simulink model "rfsoc4x2_ospfb_128"  (R2021a)
(part 2 of 221)

      mask Callback t224_QT_adc3_enable: enable_adc_opt(gcb,224,3,'QT');
      mask TypeOptions t224_QT_adc3_digital_output: Real | I/Q
      mask Callback t224_QT_adc3_digital_output:
      | validate_digital_data(gcb,224,3,'QT');
      | update_axis_clk(gcb,224);
      mask TypeOptions t224_QT_adc3_dec_mode: 1x | 2x | 3x | 4x | 5x | 6x | 8x | 10x | 12x | 16x | 20x | 24x | 40x
      mask Callback t224_QT_adc3_dec_mode: update_axis_clk(gcb,224);
      mask TypeOptions t224_QT_adc3_sample_per_cycle: 4 | 5 | 6 | 7 | 8 | 9 | 10 | 11 | 12
      mask Callback t224_QT_adc3_sample_per_cycle: update_axis_clk_label(gcb,224);
      mask TypeOptions t224_QT_adc3_mixer_type: Bypassed
      mask Callback t224_QT_adc3_mixer_type: mixertype_callback(gcb,224,3,'QT');
      mask TypeOptions t224_QT_adc3_mixer_mode: Real -> Real
      mask Callback t224_QT_adc3_mixer_mode: mixer_callback(gcb,224,3,'QT')
      mask TypeOptions t224_QT_adc3_coarse_freq: 0
      mask TypeOptions t224_QT_adc3_nyquist_zone: Zone 1 | Zone 2
      mask TypeOptions t224_QT_adc3_cal_mode: Mode 1 | Mode 2
      mask Callback t224_DT_adc0_enable: enable_adc_opt(gcb,224,0,'DT');
      mask TypeOptions t224_DT_adc0_digital_output: Real | I/Q
      mask Callback t224_DT_adc0_digital_output:
      | validate_digital_data(gcb,224,0,'DT');
      | update_axis_clk(gcb,224);
      mask TypeOptions t224_DT_adc0_dec_mode: 1x | 2x | 3x | 4x | 5x | 6x | 8x | 10x | 12x | 16x | 20x | 24x | 40x
      mask Callback t224_DT_adc0_dec_mode:
      | % if I/Q output mode, need to copy interp factor before updating axis clk
      | % note only the even slice for the tile makes this check
      | if chk_param(gcb, 't224_DT_adc0_mixer_mode', 'I/Q -> I/Q')
      |   dec_mode = get_param(gcb, 't224_DT_adc0_dec_mode');
      |   set_param(gcb, 't224_DT_adc1_dec_mode', dec_mode);
      | end
      | 
      | update_axis_clk(gcb,224);
      mask TypeOptions t224_DT_adc0_sample_per_cycle: 4 | 5 | 6 | 7 | 8 | 9 | 10 | 11 | 12
      mask Callback t224_DT_adc0_sample_per_cycle:
      | % if I/Q output mode, need to copy samples per clk before updating axis clk
      | % note only the even slice for the tile makes this check
      | if chk_param(gcb, 't224_DT_adc0_mixer_mode', 'I/Q -> I/Q')
      |   spc = get_param(gcb, 't224_DT_adc0_sample_per_cycle');
      |   set_param(gcb, 't224_DT_adc1_sample_per_cycle', spc);
      | end
      | update_axis_clk_label(gcb,224);
      mask TypeOptions t224_DT_adc0_mixer_type: Bypassed
      mask Callback t224_DT_adc0_mixer_type: mixertype_callback(gcb,224,0,'DT');
      mask TypeOptions t224_DT_adc0_mixer_mode: Real -> Real
      mask Callback t224_DT_adc0_mixer_mode: mixer_callback(gcb,224,0,'DT');
      mask TypeOptions t224_DT_adc0_coarse_freq: 0
      mask TypeOptions t224_DT_adc0_nyquist_zone: Zone 1 | Zone 2
      mask TypeOptions t224_DT_adc0_cal_mode: Mode 1 | Mode 2
      mask Callback t224_DT_adc1_enable: enable_adc_opt(gcb,224,1,'DT');
      mask TypeOptions t224_DT_adc1_digital_output: Real | I/Q
      mask Callback t224_DT_adc1_digital_output:
      | validate_digital_data(gcb,224,1,'DT');
      | update_axis_clk(gcb,224);
      mask TypeOptions t224_DT_adc1_dec_mode: 1x | 2x | 3x | 4x | 5x | 6x | 8x | 10x | 12x | 16x | 20x | 24x | 40x
      mask Callback t224_DT_adc1_dec_mode: update_axis_clk(gcb,224);
      mask TypeOptions t224_DT_adc1_sample_per_cycle: 4 | 5 | 6 | 7 | 8 | 9 | 10 | 11 | 12
      mask Callback t224_DT_adc1_sample_per_cycle:
      | %update_axis_clk(gcb);
      | update_axis_clk_label(gcb,224);
      mask TypeOptions t224_DT_adc1_mixer_type: Bypassed
      mask Callback t224_DT_adc1_mixer_type: mixertype_callback(gcb,224,1,'DT');
      mask TypeOptions t224_DT_adc1_mixer_mode: Real -> Real
      mask Callback t224_DT_adc1_mixer_mode: mixer_callback(gcb,224,1,'DT');
      mask TypeOptions t224_DT_adc1_coarse_freq: 0
      mask TypeOptions t224_DT_adc1_nyquist_zone: Zone 1 | Zone 2
      mask TypeOptions t224_DT_adc1_cal_mode: Mode 1 | Mode 2
      mask Callback t225_sample_rate: update_rfdc_clocking(gcb,225);
      mask TypeOptions t225_clk_out: 100 | 50 | 25 | 12.5
      mask Callback t225_enable_pll:
      | %update_rfdc_clocking(gcb);
      | update_pll(gcb,225);
      mask TypeOptions t225_ref_clk: 738.462 | 685.714 | 640 | 600 | 564.706 | 533.333 | 505.263 | 480 | 457.143 | 436.364 | 417.391 | 400 | 384 | 369.231 | 355.556 | 342.857 | 331.034 | 320 | 309.677 | 300 | 290.909 | 282.353 | 274.286 | 266.667 | 259.459 | 252.632 | 246.154 | 240 | 234.146 | 228.571 | 223.256 | 218.182 | 213.333 | 208.696 | 204.255 | 200 | 195.918 | 192 | 188.235 | 184.615 | 181.132 | 177.778 | 174.545 | 171.429 | 168.421 | 165.517 | 162.712 | 160 | 157.377 | 154.839 | 152.381 | 150 | 147.692 | 145.455 | 143.284 | 141.176 | 139.13 | 137.143 | 135.211 | 133.333 | 131.507 | 129.73 | 128 | 126.316 | 124.675 | 123.077 | 121.519 | 120 | 118.519 | 117.073 | 115.663 | 114.286 | 112.941 | 111.628 | 110.345 | 109.091 | 107.865 | 106.667 | 105.495 | 104.348 | 103.226
      mask Callback t225_QT_adc0_enable: enable_adc_opt(gcb,225,0,'QT');
      mask TypeOptions t225_QT_adc0_digital_output: Real | I/Q
      mask Callback t225_QT_adc0_digital_output:
      | validate_digital_data(gcb,225,0,'QT');
      | update_axis_clk(gcb,225);
      mask TypeOptions t225_QT_adc0_dec_mode: 1x | 2x | 3x | 4x | 5x | 6x | 8x | 10x | 12x | 16x | 20x | 24x | 40x
      mask Callback t225_QT_adc0_dec_mode:
      | % if I/Q output mode, need to copy interp factor before updating axis clk
      | % note only the even slice for the tile makes this check
      | if chk_param(gcb, 't225_QT_adc0_mixer_mode', 'I/Q -> I/Q')
      |   dec_mode = get_param(gcb, 't225_QT_adc0_dec_mode');
      |   set_param(gcb, 't225_QT_adc1_dec_mode', dec_mode);
      | end
      | update_axis_clk(gcb,225);
      mask TypeOptions t225_QT_adc0_sample_per_cycle: 4 | 5 | 6 | 7 | 8 | 9 | 10 | 11 | 12
      mask Callback t225_QT_adc0_sample_per_cycle:
      | % if I/Q output mode, need to copy samples per clk before updating axis clk
      | % note only the even slice for the tile makes this check
      | if chk_param(gcb, 't225_QT_adc0_mixer_mode', 'I/Q -> I/Q')
      |   spc = get_param(gcb, 't225_QT_adc0_sample_per_cycle');
      |   set_param(gcb, 't225_QT_adc1_sample_per_cycle', spc);
      | end
      | update_axis_clk_label(gcb,225);
      mask TypeOptions t225_QT_adc0_mixer_type: Bypassed
      mask Callback t225_QT_adc0_mixer_type: mixertype_callback(gcb,225,0,'QT');
      mask TypeOptions t225_QT_adc0_mixer_mode: Real -> Real
      mask Callback t225_QT_adc0_mixer_mode: mixer_callback(gcb,225,0,'QT');
      mask TypeOptions t225_QT_adc0_coarse_freq: 0
      mask TypeOptions t225_QT_adc0_nyquist_zone: Zone 1 | Zone 2
      mask TypeOptions t225_QT_adc0_cal_mode: Mode 1 | Mode 2
      mask Callback t225_QT_adc1_enable: enable_adc_opt(gcb,225,1,'QT');
      mask TypeOptions t225_QT_adc1_digital_output: Real | I/Q
      mask Callback t225_QT_adc1_digital_output:
      | validate_digital_data(gcb,225,1,'QT');
      | update_axis_clk(gcb,225);
      mask TypeOptions t225_QT_adc1_dec_mode: 1x | 2x | 3x | 4x | 5x | 6x | 8x | 10x | 12x | 16x | 20x | 24x | 40x
      mask Callback t225_QT_adc1_dec_mode: update_axis_clk(gcb,225);
      mask TypeOptions t225_QT_adc1_sample_per_cycle: 4 | 5 | 6 | 7 | 8 | 9 | 10 | 11 | 12
      mask Callback t225_QT_adc1_sample_per_cycle: update_axis_clk_label(gcb,225);
      mask TypeOptions t225_QT_adc1_mixer_type: Bypassed
      mask Callback t225_QT_adc1_mixer_type: mixertype_callback(gcb,225,1,'QT');
      mask TypeOptions t225_QT_adc1_mixer_mode: Real -> Real
      mask Callback t225_QT_adc1_mixer_mode: mixer_callback(gcb,225,1,'QT')
      mask TypeOptions t225_QT_adc1_coarse_freq: 0
      mask TypeOptions t225_QT_adc1_nyquist_zone: Zone 1 | Zone 2
      mask TypeOptions t225_QT_adc1_cal_mode: Mode 1 | Mode 2
      mask Callback t225_QT_adc2_enable: enable_adc_opt(gcb,225,2,'QT');
      mask TypeOptions t225_QT_adc2_digital_output: Real | I/Q
      mask Callback t225_QT_adc2_digital_output:
      | validate_digital_data(gcb,225,2,'QT');
      | update_axis_clk(gcb,225);
      mask TypeOptions t225_QT_adc2_dec_mode: 1x | 2x | 3x | 4x | 5x | 6x | 8x | 10x | 12x | 16x | 20x | 24x | 40x
      mask Callback t225_QT_adc2_dec_mode:
      | % if I/Q output mode, need to copy interp factor before updating axis clk
      | % note only the even slice for the tile makes this check
      | if chk_param(gcb, 't225_QT_adc2_mixer_mode', 'I/Q -> I/Q')
      |   dec_mode = get_param(gcb, 't225_QT_adc2_dec_mode');
      |   set_param(gcb, 't225_QT_adc3_dec_mode', dec_mode);
      | end
      | update_axis_clk(gcb,225);
      mask TypeOptions t225_QT_adc2_sample_per_cycle: 4 | 5 | 6 | 7 | 8 | 9 | 10 | 11 | 12
      mask Callback t225_QT_adc2_sample_per_cycle:
      | % if I/Q output mode, need to copy samples per clk before updating axis clk
      | % note only the even slice for the tile makes this check
      | if chk_param(gcb, 't225_QT_adc2_mixer_mode', 'I/Q -> I/Q')
      |   spc = get_param(gcb, 't225_QT_adc2_sample_per_cycle');
      |   set_param(gcb, 't225_QT_adc3_sample_per_cycle', spc);
      | end
      | update_axis_clk_label(gcb,225);
      mask TypeOptions t225_QT_adc2_mixer_type: Bypassed
      mask Callback t225_QT_adc2_mixer_type: mixertype_callback(gcb,225,2,'QT');
      mask TypeOptions t225_QT_adc2_mixer_mode: Real -> Real
      mask Callback t225_QT_adc2_mixer_mode: mixer_callback(gcb,225,2,'QT')
      mask TypeOptions t225_QT_adc2_coarse_freq: 0
      mask TypeOptions t225_QT_adc2_nyquist_zone: Zone 1 | Zone 2
      mask TypeOptions t225_QT_adc2_cal_mode: Mode 1 | Mode 2
      mask Callback t225_QT_adc3_enable: enable_adc_opt(gcb,225,3,'QT');
      mask TypeOptions t225_QT_adc3_digital_output: Real | I/Q
      mask Callback t225_QT_adc3_digital_output:
      | validate_digital_data(gcb,225,3,'QT');
      | update_axis_clk(gcb,225);
      mask TypeOptions t225_QT_adc3_dec_mode: 1x | 2x | 3x | 4x | 5x | 6x | 8x | 10x | 12x | 16x | 20x | 24x | 40x
      mask Callback t225_QT_adc3_dec_mode: update_axis_clk(gcb,225);
      mask TypeOptions t225_QT_adc3_sample_per_cycle: 4 | 5 | 6 | 7 | 8 | 9 | 10 | 11 | 12
      mask Callback t225_QT_adc3_sample_per_cycle: update_axis_clk_label(gcb,225);
      mask TypeOptions t225_QT_adc3_mixer_type: Bypassed
      mask Callback t225_QT_adc3_mixer_type: mixertype_callback(gcb,225,3,'QT');
      mask TypeOptions t225_QT_adc3_mixer_mode: Real -> Real
      mask Callback t225_QT_adc3_mixer_mode: mixer_callback(gcb,225,3,'QT')
      mask TypeOptions t225_QT_adc3_coarse_freq: 0
      mask TypeOptions t225_QT_adc3_nyquist_zone: Zone 1 | Zone 2
      mask TypeOptions t225_QT_adc3_cal_mode: Mode 1 | Mode 2
      mask Callback t225_DT_adc0_enable: enable_adc_opt(gcb,225,0,'DT');
      mask TypeOptions t225_DT_adc0_digital_output: Real | I/Q
      mask Callback t225_DT_adc0_digital_output:
      | validate_digital_data(gcb,225,0,'DT');
      | update_axis_clk(gcb,225);
      mask TypeOptions t225_DT_adc0_dec_mode: 1x | 2x | 3x | 4x | 5x | 6x | 8x | 10x | 12x | 16x | 20x | 24x | 40x
      mask Callback t225_DT_adc0_dec_mode:
      | % if I/Q output mode, need to copy interp factor before updating axis clk
      | % note only the even slice for the tile makes this check
      | if chk_param(gcb, 't225_DT_adc0_mixer_mode', 'I/Q -> I/Q')
      |   dec_mode = get_param(gcb, 't225_DT_adc0_dec_mode');
      |   set_param(gcb, 't225_DT_adc1_dec_mode', dec_mode);
      | end
      | update_axis_clk(gcb,225);
      mask TypeOptions t225_DT_adc0_sample_per_cycle: 4 | 5 | 6 | 7 | 8 | 9 | 10 | 11 | 12
      mask Callback t225_DT_adc0_sample_per_cycle:
      | % if I/Q output mode, need to copy samples per clk before updating axis clk
      | % note only the even slice for the tile makes this check
      | if chk_param(gcb, 't225_DT_adc0_mixer_mode', 'I/Q -> I/Q')
      |   spc = get_param(gcb, 't225_DT_adc0_sample_per_cycle');
      |   set_param(gcb, 't225_DT_adc1_sample_per_cycle', spc);
      | end
      | update_axis_clk_label(gcb,225);
      mask TypeOptions t225_DT_adc0_mixer_type: Bypassed
      mask Callback t225_DT_adc0_mixer_type: mixertype_callback(gcb,225,0,'DT');
      mask TypeOptions t225_DT_adc0_mixer_mode: Real -> Real
      mask Callback t225_DT_adc0_mixer_mode: mixer_callback(gcb,225,0,'DT');
      mask TypeOptions t225_DT_adc0_coarse_freq: 0
      mask TypeOptions t225_DT_adc0_nyquist_zone: Zone 1 | Zone 2
      mask TypeOptions t225_DT_adc0_cal_mode: Mode 1 | Mode 2
      mask Callback t225_DT_adc1_enable: enable_adc_opt(gcb,225,1,'DT');
      mask TypeOptions t225_DT_adc1_digital_output: Real | I/Q
      mask Callback t225_DT_adc1_digital_output:
      | validate_digital_data(gcb,225,1,'DT');
      | update_axis_clk(gcb,225);
      mask TypeOptions t225_DT_adc1_dec_mode: 1x | 2x | 3x | 4x | 5x | 6x | 8x | 10x | 12x | 16x | 20x | 24x | 40x
      mask Callback t225_DT_adc1_dec_mode: update_axis_clk(gcb,225);
      mask TypeOptions t225_DT_adc1_sample_per_cycle: 4 | 5 | 6 | 7 | 8 | 9 | 10 | 11 | 12
      mask Callback t225_DT_adc1_sample_per_cycle:
      | %update_axis_clk(gcb);
      | update_axis_clk_label(gcb,225);
      mask TypeOptions t225_DT_adc1_mixer_type: Bypassed
      mask Callback t225_DT_adc1_mixer_type: mixertype_callback(gcb,225,1,'DT');
      mask TypeOptions t225_DT_adc1_mixer_mode: Real -> Real
      mask Callback t225_DT_adc1_mixer_mode: mixer_callback(gcb,225,1,'DT');
      mask TypeOptions t225_DT_adc1_coarse_freq: 0
      mask TypeOptions t225_DT_adc1_nyquist_zone: Zone 1 | Zone 2
      mask TypeOptions t225_DT_adc1_cal_mode: Mode 1 | Mode 2
      mask Callback t226_sample_rate: update_rfdc_clocking(gcb,226);
      mask TypeOptions t226_clk_out: 100 | 50 | 25 | 12.5
      mask Callback t226_enable_pll:
      | %update_rfdc_clocking(gcb);
      | update_pll(gcb,226);
      mask TypeOptions t226_ref_clk: 738.462 | 685.714 | 640 | 600 | 564.706 | 533.333 | 505.263 | 480 | 457.143 | 436.364 | 417.391 | 400 | 384 | 369.231 | 355.556 | 342.857 | 331.034 | 320 | 309.677 | 300 | 290.909 | 282.353 | 274.286 | 266.667 | 259.459 | 252.632 | 246.154 | 240 | 234.146 | 228.571 | 223.256 | 218.182 | 213.333 | 208.696 | 204.255 | 200 | 195.918 | 192 | 188.235 | 184.615 | 181.132 | 177.778 | 174.545 | 171.429 | 168.421 | 165.517 | 162.712 | 160 | 157.377 | 154.839 | 152.381 | 150 | 147.692 | 145.455 | 143.284 | 141.176 | 139.13 | 137.143 | 135.211 | 133.333 | 131.507 | 129.73 | 128 | 126.316 | 124.675 | 123.077 | 121.519 | 120 | 118.519 | 117.073 | 115.663 | 114.286 | 112.941 | 111.628 | 110.345 | 109.091 | 107.865 | 106.667 | 105.495 | 104.348 | 103.226
      mask Callback t226_QT_adc0_enable: enable_adc_opt(gcb,226,0,'QT');
      mask TypeOptions t226_QT_adc0_digital_output: Real | I/Q
      mask Callback t226_QT_adc0_digital_output:
      | validate_digital_data(gcb,226,0,'QT');
      | update_axis_clk(gcb,226);
      mask TypeOptions t226_QT_adc0_dec_mode: 1x | 2x | 3x | 4x | 5x | 6x | 8x | 10x | 12x | 16x | 20x | 24x | 40x
      mask Callback t226_QT_adc0_dec_mode:
      | % if I/Q output mode, need to copy interp factor before updating axis clk
      | % note only the even slice for the tile makes this check
      | if chk_param(gcb, 't226_QT_adc0_mixer_mode', 'I/Q -> I/Q')
      |   dec_mode = get_param(gcb, 't226_QT_adc0_dec_mode');
      |   set_param(gcb, 't226_QT_adc1_dec_mode', dec_mode);
      | end
      | update_axis_clk(gcb,226);
      mask TypeOptions t226_QT_adc0_sample_per_cycle: 4 | 5 | 6 | 7 | 8 | 9 | 10 | 11 | 12
      mask Callback t226_QT_adc0_sample_per_cycle:
      | % if I/Q output mode, need to copy samples per clk before updating axis clk
      | % note only the even slice for the tile makes this check
      | if chk_param(gcb, 't226_QT_adc0_mixer_mode', 'I/Q -> I/Q')
      |   spc = get_param(gcb, 't226_QT_adc0_sample_per_cycle');
      |   set_param(gcb, 't226_QT_adc1_sample_per_cycle', spc);
      | end
      | update_axis_clk_label(gcb,226);
      mask TypeOptions t226_QT_adc0_mixer_type: Bypassed
      mask Callback t226_QT_adc0_mixer_type: mixertype_callback(gcb,226,0,'QT');
      mask TypeOptions t226_QT_adc0_mixer_mode: Real -> Real
      mask Callback t226_QT_adc0_mixer_mode: mixer_callback(gcb,226,0,'QT');
      mask TypeOptions t226_QT_adc0_coarse_freq: 0
      mask TypeOptions t226_QT_adc0_nyquist_zone: Zone 1 | Zone 2
      mask TypeOptions t226_QT_adc0_cal_mode: Mode 1 | Mode 2
      mask Callback t226_QT_adc1_enable: enable_adc_opt(gcb,226,1,'QT');
      mask TypeOptions t226_QT_adc1_digital_output: Real | I/Q
      mask Callback t226_QT_adc1_digital_output:
      | validate_digital_data(gcb,226,1,'QT');
      | update_axis_clk(gcb,226);
      mask TypeOptions t226_QT_adc1_dec_mode: 1x | 2x | 3x | 4x | 5x | 6x | 8x | 10x | 12x | 16x | 20x | 24x | 40x
      mask Callback t226_QT_adc1_dec_mode: update_axis_clk(gcb,226);
      mask TypeOptions t226_QT_adc1_sample_per_cycle: 4 | 5 | 6 | 7 | 8 | 9 | 10 | 11 | 12
      mask Callback t226_QT_adc1_sample_per_cycle: update_axis_clk_label(gcb,226);
      mask TypeOptions t226_QT_adc1_mixer_type: Bypassed
      mask Callback t226_QT_adc1_mixer_type: mixertype_callback(gcb,226,1,'QT');
      mask TypeOptions t226_QT_adc1_mixer_mode: Real -> Real
      mask Callback t226_QT_adc1_mixer_mode: mixer_callback(gcb,226,1,'QT')
      mask TypeOptions t226_QT_adc1_coarse_freq: 0
      mask TypeOptions t226_QT_adc1_nyquist_zone: Zone 1 | Zone 2
      mask TypeOptions t226_QT_adc1_cal_mode: Mode 1 | Mode 2
      mask Callback t226_QT_adc2_enable: enable_adc_opt(gcb,226,2,'QT');
      mask TypeOptions t226_QT_adc2_digital_output: Real | I/Q
      mask Callback t226_QT_adc2_digital_output:
      | validate_digital_data(gcb,226,2,'QT');
      | update_axis_clk(gcb,226);
      mask TypeOptions t226_QT_adc2_dec_mode: 1x | 2x | 3x | 4x | 5x | 6x | 8x | 10x | 12x | 16x | 20x | 24x | 40x
      mask Callback t226_QT_adc2_dec_mode:
      | % if I/Q output mode, need to copy interp factor before updating axis clk
      | % note only the even slice for the tile makes this check
      | if chk_param(gcb, 't226_QT_adc2_mixer_mode', 'I/Q -> I/Q')
      |   dec_mode = get_param(gcb, 't226_QT_adc2_dec_mode');
      |   set_param(gcb, 't226_QT_adc3_dec_mode', dec_mode);
      | end
      | update_axis_clk(gcb,226);
      mask TypeOptions t226_QT_adc2_sample_per_cycle: 4 | 5 | 6 | 7 | 8 | 9 | 10 | 11 | 12
      mask Callback t226_QT_adc2_sample_per_cycle:
      | % if I/Q output mode, need to copy samples per clk before updating axis clk
      | % note only the even slice for the tile makes this check
      | if chk_param(gcb, 't226_QT_adc2_mixer_mode', 'I/Q -> I/Q')
      |   spc = get_param(gcb, 't226_QT_adc2_sample_per_cycle');
      |   set_param(gcb, 't226_QT_adc3_sample_per_cycle', spc);
      | end
      | update_axis_clk_label(gcb,226);
      mask TypeOptions t226_QT_adc2_mixer_type: Bypassed
      mask Callback t226_QT_adc2_mixer_type: mixertype_callback(gcb,226,2,'QT');
      mask TypeOptions t226_QT_adc2_mixer_mode: Real -> Real
      mask Callback t226_QT_adc2_mixer_mode: mixer_callback(gcb,226,2,'QT')
      mask TypeOptions t226_QT_adc2_coarse_freq: 0
      mask TypeOptions t226_QT_adc2_nyquist_zone: Zone 1 | Zone 2
      mask TypeOptions t226_QT_adc2_cal_mode: Mode 1 | Mode 2
      mask Callback t226_QT_adc3_enable: enable_adc_opt(gcb,226,3,'QT');
      mask TypeOptions t226_QT_adc3_digital_output: Real | I/Q
      mask Callback t226_QT_adc3_digital_output:
      | validate_digital_data(gcb,226,3,'QT');
      | update_axis_clk(gcb,226);
      mask TypeOptions t226_QT_adc3_dec_mode: 1x | 2x | 3x | 4x | 5x | 6x | 8x | 10x | 12x | 16x | 20x | 24x | 40x
      mask Callback t226_QT_adc3_dec_mode: update_axis_clk(gcb,226);
      mask TypeOptions t226_QT_adc3_sample_per_cycle: 4 | 5 | 6 | 7 | 8 | 9 | 10 | 11 | 12
      mask Callback t226_QT_adc3_sample_per_cycle: update_axis_clk_label(gcb,226);
      mask TypeOptions t226_QT_adc3_mixer_type: Bypassed
      mask Callback t226_QT_adc3_mixer_type: mixertype_callback(gcb,226,3,'QT');
      mask TypeOptions t226_QT_adc3_mixer_mode: Real -> Real
      mask Callback t226_QT_adc3_mixer_mode: mixer_callback(gcb,226,3,'QT')
      mask TypeOptions t226_QT_adc3_coarse_freq: 0
      mask TypeOptions t226_QT_adc3_nyquist_zone: Zone 1 | Zone 2
      mask TypeOptions t226_QT_adc3_cal_mode: Mode 1 | Mode 2
      mask Callback t226_DT_adc0_enable: enable_adc_opt(gcb,226,0,'DT');
      mask TypeOptions t226_DT_adc0_digital_output: Real | I/Q
      mask Callback t226_DT_adc0_digital_output:
      | validate_digital_data(gcb,226,0,'DT');
      | update_axis_clk(gcb,226);
      mask TypeOptions t226_DT_adc0_dec_mode: 1x | 2x | 3x | 4x | 5x | 6x | 8x | 10x | 12x | 16x | 20x | 24x | 40x
      mask Callback t226_DT_adc0_dec_mode:
      | % if I/Q output mode, need to copy interp factor before updating axis clk
      | % note only the even slice for the tile makes this check
      | if chk_param(gcb, 't226_DT_adc0_mixer_mode', 'I/Q -> I/Q')
      |   dec_mode = get_param(gcb, 't226_DT_adc0_dec_mode');
      |   set_param(gcb, 't226_DT_adc1_dec_mode', dec_mode);
      | end
      | update_axis_clk(gcb,226);
      mask TypeOptions t226_DT_adc0_sample_per_cycle: 4 | 5 | 6 | 7 | 8 | 9 | 10 | 11 | 12
      mask Callback t226_DT_adc0_sample_per_cycle:
      | % if I/Q output mode, need to copy samples per clk before updating axis clk
      | % note only the even slice for the tile makes this check
      | if chk_param(gcb, 't226_DT_adc0_mixer_mode', 'I/Q -> I/Q')
      |   spc = get_param(gcb, 't226_DT_adc0_sample_per_cycle');
      |   set_param(gcb, 't226_DT_adc1_sample_per_cycle', spc);
      | end
      | update_axis_clk_label(gcb,226);
      mask TypeOptions t226_DT_adc0_mixer_type: Bypassed
      mask Callback t226_DT_adc0_mixer_type: mixertype_callback(gcb,226,0,'DT');
      mask TypeOptions t226_DT_adc0_mixer_mode: Real -> Real
      mask Callback t226_DT_adc0_mixer_mode: mixer_callback(gcb,226,0,'DT');
      mask TypeOptions t226_DT_adc0_coarse_freq: 0
      mask TypeOptions t226_DT_adc0_nyquist_zone: Zone 1 | Zone 2
      mask TypeOptions t226_DT_adc0_cal_mode: Mode 1 | Mode 2
      mask Callback t226_DT_adc1_enable: enable_adc_opt(gcb,226,1,'DT');
      mask TypeOptions t226_DT_adc1_digital_output: Real | I/Q
      mask Callback t226_DT_adc1_digital_output:
      | validate_digital_data(gcb,226,1,'DT');
      | update_axis_clk(gcb,226);
      mask TypeOptions t226_DT_adc1_dec_mode: 1x | 2x | 3x | 4x | 5x | 6x | 8x | 10x | 12x | 16x | 20x | 24x | 40x
      mask Callback t226_DT_adc1_dec_mode: update_axis_clk(gcb,226);
      mask TypeOptions t226_DT_adc1_sample_per_cycle: 4 | 5 | 6 | 7 | 8 | 9 | 10 | 11 | 12
      mask Callback t226_DT_adc1_sample_per_cycle:
      | %update_axis_clk(gcb);
      | update_axis_clk_label(gcb,226);
      mask TypeOptions t226_DT_adc1_mixer_type: Bypassed
      mask Callback t226_DT_adc1_mixer_type: mixertype_callback(gcb,226,1,'DT');
      mask TypeOptions t226_DT_adc1_mixer_mode: Real -> Real
      mask Callback t226_DT_adc1_mixer_mode: mixer_callback(gcb,226,1,'DT');
      mask TypeOptions t226_DT_adc1_coarse_freq: 0
      mask TypeOptions t226_DT_adc1_nyquist_zone: Zone 1 | Zone 2
      mask TypeOptions t226_DT_adc1_cal_mode: Mode 1 | Mode 2
      mask Callback t227_sample_rate: update_rfdc_clocking(gcb,227);
      mask TypeOptions t227_clk_out: 100 | 50 | 25 | 12.5
      mask Callback t227_enable_pll:
      | %update_rfdc_clocking(gcb);
      | update_pll(gcb,227);
      mask TypeOptions t227_ref_clk: 738.462 | 685.714 | 640 | 600 | 564.706 | 533.333 | 505.263 | 480 | 457.143 | 436.364 | 417.391 | 400 | 384 | 369.231 | 355.556 | 342.857 | 331.034 | 320 | 309.677 | 300 | 290.909 | 282.353 | 274.286 | 266.667 | 259.459 | 252.632 | 246.154 | 240 | 234.146 | 228.571 | 223.256 | 218.182 | 213.333 | 208.696 | 204.255 | 200 | 195.918 | 192 | 188.235 | 184.615 | 181.132 | 177.778 | 174.545 | 171.429 | 168.421 | 165.517 | 162.712 | 160 | 157.377 | 154.839 | 152.381 | 150 | 147.692 | 145.455 | 143.284 | 141.176 | 139.13 | 137.143 | 135.211 | 133.333 | 131.507 | 129.73 | 128 | 126.316 | 124.675 | 123.077 | 121.519 | 120 | 118.519 | 117.073 | 115.663 | 114.286 | 112.941 | 111.628 | 110.345 | 109.091 | 107.865 | 106.667 | 105.495 | 104.348 | 103.226
      mask Callback t227_QT_adc0_enable: enable_adc_opt(gcb,227,0,'QT');
      mask TypeOptions t227_QT_adc0_digital_output: Real | I/Q
      mask Callback t227_QT_adc0_digital_output:
      | validate_digital_data(gcb,227,0,'QT');
      | update_axis_clk(gcb,227);
      mask TypeOptions t227_QT_adc0_dec_mode: 1x | 2x | 3x | 4x | 5x | 6x | 8x | 10x | 12x | 16x | 20x | 24x | 40x
      mask Callback t227_QT_adc0_dec_mode:
      | % if I/Q output mode, need to copy interp factor before updating axis clk
      | % note only the even slice for the tile makes this check
      | if chk_param(gcb, 't227_QT_adc0_mixer_mode', 'I/Q -> I/Q')
      |   dec_mode = get_param(gcb, 't227_QT_adc0_dec_mode');
      |   set_param(gcb, 't227_QT_adc1_dec_mode', dec_mode);
      | end
      | update_axis_clk(gcb,227);
      mask TypeOptions t227_QT_adc0_sample_per_cycle: 4 | 5 | 6 | 7 | 8 | 9 | 10 | 11 | 12
      mask Callback t227_QT_adc0_sample_per_cycle:
      | % if I/Q output mode, need to copy samples per clk before updating axis clk
      | % note only the even slice for the tile makes this check
      | if chk_param(gcb, 't227_QT_adc0_mixer_mode', 'I/Q -> I/Q')
      |   spc = get_param(gcb, 't227_QT_adc0_sample_per_cycle');
      |   set_param(gcb, 't227_QT_adc1_sample_per_cycle', spc);
      | end
      | update_axis_clk_label(gcb,227);
      mask TypeOptions t227_QT_adc0_mixer_type: Bypassed
      mask Callback t227_QT_adc0_mixer_type: mixertype_callback(gcb,227,0,'QT');
      mask TypeOptions t227_QT_adc0_mixer_mode: Real -> Real
      mask Callback t227_QT_adc0_mixer_mode: mixer_callback(gcb,227,0,'QT');
      mask TypeOptions t227_QT_adc0_coarse_freq: 0
      mask TypeOptions t227_QT_adc0_nyquist_zone: Zone 1 | Zone 2
      mask TypeOptions t227_QT_adc0_cal_mode: Mode 1 | Mode 2
      mask Callback t227_QT_adc1_enable: enable_adc_opt(gcb,227,1,'QT');
      mask TypeOptions t227_QT_adc1_digital_output: Real | I/Q
      mask Callback t227_QT_adc1_digital_output:
      | validate_digital_data(gcb,227,1,'QT');
      | update_axis_clk(gcb,227);
      mask TypeOptions t227_QT_adc1_dec_mode: 1x | 2x | 3x | 4x | 5x | 6x | 8x | 10x | 12x | 16x | 20x | 24x | 40x
      mask Callback t227_QT_adc1_dec_mode: update_axis_clk(gcb,227);
      mask TypeOptions t227_QT_adc1_sample_per_cycle: 4 | 5 | 6 | 7 | 8 | 9 | 10 | 11 | 12
      mask Callback t227_QT_adc1_sample_per_cycle: update_axis_clk_label(gcb,227);
      mask TypeOptions t227_QT_adc1_mixer_type: Bypassed
      mask Callback t227_QT_adc1_mixer_type: mixertype_callback(gcb,227,1,'QT');
      mask TypeOptions t227_QT_adc1_mixer_mode: Real -> Real
      mask Callback t227_QT_adc1_mixer_mode: mixer_callback(gcb,227,1,'QT')
      mask TypeOptions t227_QT_adc1_coarse_freq: 0
      mask TypeOptions t227_QT_adc1_nyquist_zone: Zone 1 | Zone 2
      mask TypeOptions t227_QT_adc1_cal_mode: Mode 1 | Mode 2
      mask Callback t227_QT_adc2_enable: enable_adc_opt(gcb,227,2,'QT');
      mask TypeOptions t227_QT_adc2_digital_output: Real | I/Q
      mask Callback t227_QT_adc2_digital_output:
      | validate_digital_data(gcb,227,2,'QT');
      | update_axis_clk(gcb,227);
      mask TypeOptions t227_QT_adc2_dec_mode: 1x | 2x | 3x | 4x | 5x | 6x | 8x | 10x | 12x | 16x | 20x | 24x | 40x
      mask Callback t227_QT_adc2_dec_mode:
      | % if I/Q output mode, need to copy interp factor before updating axis clk
      | % note only the even slice for the tile makes this check
      | if chk_param(gcb, 't227_QT_adc2_mixer_mode', 'I/Q -> I/Q')
      |   dec_mode = get_param(gcb, 't227_QT_adc2_dec_mode');
      |   set_param(gcb, 't227_QT_adc3_dec_mode', dec_mode);
      | end
      | update_axis_clk(gcb,227);
      mask TypeOptions t227_QT_adc2_sample_per_cycle: 4 | 5 | 6 | 7 | 8 | 9 | 10 | 11 | 12
      mask Callback t227_QT_adc2_sample_per_cycle:
      | % if I/Q output mode, need to copy samples per clk before updating axis clk
      | % note only the even slice for the tile makes this check
      | if chk_param(gcb, 't227_QT_adc2_mixer_mode', 'I/Q -> I/Q')
      |   spc = get_param(gcb, 't227_QT_adc2_sample_per_cycle');
      |   set_param(gcb, 't227_QT_adc3_sample_per_cycle', spc);
      | end
      | update_axis_clk_label(gcb,227);
      mask TypeOptions t227_QT_adc2_mixer_type: Bypassed
      mask Callback t227_QT_adc2_mixer_type: mixertype_callback(gcb,227,2,'QT');
      mask TypeOptions t227_QT_adc2_mixer_mode: Real -> Real
      mask Callback t227_QT_adc2_mixer_mode: mixer_callback(gcb,227,2,'QT')
      mask TypeOptions t227_QT_adc2_coarse_freq: 0
      mask TypeOptions t227_QT_adc2_nyquist_zone: Zone 1 | Zone 2
      mask TypeOptions t227_QT_adc2_cal_mode: Mode 1 | Mode 2
      mask Callback t227_QT_adc3_enable: enable_adc_opt(gcb,227,3,'QT');
      mask TypeOptions t227_QT_adc3_digital_output: Real | I/Q
      mask Callback t227_QT_adc3_digital_output:
      | validate_digital_data(gcb,227,3,'QT');
      | update_axis_clk(gcb,227);
      mask TypeOptions t227_QT_adc3_dec_mode: 1x | 2x | 3x | 4x | 5x | 6x | 8x | 10x | 12x | 16x | 20x | 24x | 40x
      mask Callback t227_QT_adc3_dec_mode: update_axis_clk(gcb,227);
      mask TypeOptions t227_QT_adc3_sample_per_cycle: 4 | 5 | 6 | 7 | 8 | 9 | 10 | 11 | 12
      mask Callback t227_QT_adc3_sample_per_cycle: update_axis_clk_label(gcb,227);
      mask TypeOptions t227_QT_adc3_mixer_type: Bypassed
      mask Callback t227_QT_adc3_mixer_type: mixertype_callback(gcb,227,3,'QT');
      mask TypeOptions t227_QT_adc3_mixer_mode: Real -> Real
      mask Callback t227_QT_adc3_mixer_mode: mixer_callback(gcb,227,3,'QT')
      mask TypeOptions t227_QT_adc3_coarse_freq: 0
      mask TypeOptions t227_QT_adc3_nyquist_zone: Zone 1 | Zone 2
      mask TypeOptions t227_QT_adc3_cal_mode: Mode 1 | Mode 2
      mask Callback t227_DT_adc0_enable: enable_adc_opt(gcb,227,0,'DT');
      mask TypeOptions t227_DT_adc0_digital_output: Real | I/Q
      mask Callback t227_DT_adc0_digital_output:
      | validate_digital_data(gcb,227,0,'DT');
      | update_axis_clk(gcb,227);
      mask TypeOptions t227_DT_adc0_dec_mode: 1x | 2x | 3x | 4x | 5x | 6x | 8x | 10x | 12x | 16x | 20x | 24x | 40x
      mask Callback t227_DT_adc0_dec_mode:
      | % if I/Q output mode, need to copy interp factor before updating axis clk
      | % note only the even slice for the tile makes this check
      | if chk_param(gcb, 't227_DT_adc0_mixer_mode', 'I/Q -> I/Q')
      |   dec_mode = get_param(gcb, 't227_DT_adc0_dec_mode');
      |   set_param(gcb, 't227_DT_adc1_dec_mode', dec_mode);
      | end
      | update_axis_clk(gcb,227);
      mask TypeOptions t227_DT_adc0_sample_per_cycle: 4 | 5 | 6 | 7 | 8 | 9 | 10 | 11 | 12
      mask Callback t227_DT_adc0_sample_per_cycle:
      | % if I/Q output mode, need to copy samples per clk before updating axis clk
      | % note only the even slice for the tile makes this check
      | if chk_param(gcb, 't227_DT_adc0_mixer_mode', 'I/Q -> I/Q')
      |   spc = get_param(gcb, 't227_DT_adc0_sample_per_cycle');
      |   set_param(gcb, 't227_DT_adc1_sample_per_cycle', spc);
      | end
      | update_axis_clk_label(gcb,227);
      mask TypeOptions t227_DT_adc0_mixer_type: Bypassed
      mask Callback t227_DT_adc0_mixer_type: mixertype_callback(gcb,227,0,'DT');
      mask TypeOptions t227_DT_adc0_mixer_mode: Real -> Real
      mask Callback t227_DT_adc0_mixer_mode: mixer_callback(gcb,227,0,'DT');
      mask TypeOptions t227_DT_adc0_coarse_freq: 0
      mask TypeOptions t227_DT_adc0_nyquist_zone: Zone 1 | Zone 2
      mask TypeOptions t227_DT_adc0_cal_mode: Mode 1 | Mode 2
      mask Callback t227_DT_adc1_enable: enable_adc_opt(gcb,227,1,'DT');
      mask TypeOptions t227_DT_adc1_digital_output: Real | I/Q
      mask Callback t227_DT_adc1_digital_output:
      | validate_digital_data(gcb,227,1,'DT');
      | update_axis_clk(gcb,227);
      mask TypeOptions t227_DT_adc1_dec_mode: 1x | 2x | 3x | 4x | 5x | 6x | 8x | 10x | 12x | 16x | 20x | 24x | 40x
      mask Callback t227_DT_adc1_dec_mode: update_axis_clk(gcb,227);
      mask TypeOptions t227_DT_adc1_sample_per_cycle: 4 | 5 | 6 | 7 | 8 | 9 | 10 | 11 | 12
      mask Callback t227_DT_adc1_sample_per_cycle:
      | %update_axis_clk(gcb);
      | update_axis_clk_label(gcb,227);
      mask TypeOptions t227_DT_adc1_mixer_type: Bypassed
      mask Callback t227_DT_adc1_mixer_type: mixertype_callback(gcb,227,1,'DT');
      mask TypeOptions t227_DT_adc1_mixer_mode: Real -> Real
      mask Callback t227_DT_adc1_mixer_mode: mixer_callback(gcb,227,1,'DT');
      mask TypeOptions t227_DT_adc1_coarse_freq: 0
      mask TypeOptions t227_DT_adc1_nyquist_zone: Zone 1 | Zone 2
      mask TypeOptions t227_DT_adc1_cal_mode: Mode 1 | Mode 2
      mask Callback t228_sample_rate: update_rfdc_clocking(gcb,228);
      mask TypeOptions t228_clk_out: 125 | 62.5 | 31.25 | 15.625
      mask Callback t228_enable_pll:
      | %update_rfdc_clocking(gcb);
      | update_pll(gcb,228);
      mask TypeOptions t228_ref_clk: 2000
      mask Callback t228_QT_dac0_enable: enable_dac_opt(gcb,228,0,'QT');
      mask TypeOptions t228_QT_dac0_analog_output: Real | I/Q
      mask Callback t228_QT_dac0_analog_output:
      | validate_analog_data(gcb,228,0,'QT');
      | update_axis_clk(gcb,228);
      mask TypeOptions t228_QT_dac0_inter_mode: 1x | 2x | 3x | 4x | 5x | 6x | 8x | 10x | 12x | 16x | 20x | 24x | 40x
      mask Callback t228_QT_dac0_inter_mode:
      | % if I/Q output mode, need to copy interp factor before updating axis clk
      | % note only the even slice for the tile makes this check
      | if chk_param(gcb, 't228_QT_dac0_analog_output', 'I/Q')
      |   inter_mode = get_param(gcb, 't228_QT_dac0_inter_mode');
      |   set_param(gcb, 't228_QT_dac1_inter_mode', inter_mode);
      | end
      | 
      | update_axis_clk(gcb,228);
      mask TypeOptions t228_QT_dac0_sample_per_cycle: 4 | 5 | 6 | 7 | 8 | 9 | 10 | 11 | 12 | 13 | 14 | 15 | 16
      mask Callback t228_QT_dac0_sample_per_cycle:
      | % if I/Q output mode, need to copy samples per clk before updating axis clk
      | if chk_param(gcb, 't228_QT_dac0_analog_output', 'I/Q')
      |   spc = get_param(gcb, 't228_QT_dac0_sample_per_cycle');
      |   set_param(gcb, 't228_QT_dac1_sample_per_cycle', spc);
      | end
      | 
      | update_axis_clk_label(gcb,228);
      mask TypeOptions t228_QT_dac0_datapath_mode: DUC 0 to Fs/2 | DUC 0 to Fs/4 | DUC Fs/4 to Fs/2 | No DUC 0 to Fs/2
      mask TypeOptions t228_QT_dac0_mixer_type: Fine | Coarse
      mask Callback t228_QT_dac0_mixer_type: mixertype_callback(gcb,228,0,'QT');
      mask TypeOptions t228_QT_dac0_mixer_mode: Real -> Real | I/Q -> Real
      mask Callback t228_QT_dac0_mixer_mode: mixer_callback(gcb,228,0,'QT');
      mask TypeOptions t228_QT_dac0_coarse_freq: 0
      mask TypeOptions t228_QT_dac0_nyquist_zone: Zone 1 | Zone 2
      mask TypeOptions t228_QT_dac0_decode_mode: SNR Optimized | Linearity Optimized
      mask Callback t228_QT_dac1_enable: enable_dac_opt(gcb,228,1,'QT');
      mask TypeOptions t228_QT_dac1_analog_output: Real | I/Q
      mask Callback t228_QT_dac1_analog_output:
      | validate_analog_data(gcb,228,1,'QT');
      | update_axis_clk(gcb,228);
      mask TypeOptions t228_QT_dac1_inter_mode: 1x | 2x | 3x | 4x | 5x | 6x | 8x | 10x | 12x | 16x | 20x | 24x | 40x
      mask Callback t228_QT_dac1_inter_mode: update_axis_clk(gcb,228);
      mask TypeOptions t228_QT_dac1_sample_per_cycle: 4 | 5 | 6 | 7 | 8 | 9 | 10 | 11 | 12 | 13 | 14 | 15 | 16
      mask Callback t228_QT_dac1_sample_per_cycle: update_axis_clk_label(gcb,228);
      mask TypeOptions t228_QT_dac1_datapath_mode: DUC 0 to Fs/2 | DUC 0 to Fs/4 | DUC Fs/4 to Fs/2 | No DUC 0 to Fs/2
      mask TypeOptions t228_QT_dac1_mixer_type: Fine | Coarse
      mask Callback t228_QT_dac1_mixer_type: mixertype_callback(gcb,228,1,'QT');
      mask TypeOptions t228_QT_dac1_mixer_mode: Real -> Real | I/Q -> Real
      mask Callback t228_QT_dac1_mixer_mode: mixer_callback(gcb,228,1,'QT')
      mask TypeOptions t228_QT_dac1_coarse_freq: 0
      mask TypeOptions t228_QT_dac1_nyquist_zone: Zone 1 | Zone 2
      mask TypeOptions t228_QT_dac1_decode_mode: SNR Optimized | Linearity Optimized
      mask Callback t228_QT_dac2_enable: enable_dac_opt(gcb,228,2,'QT');
      mask TypeOptions t228_QT_dac2_analog_output: Real | I/Q
      mask Callback t228_QT_dac2_analog_output:
      | validate_analog_data(gcb,228,2,'QT');
      | update_axis_clk(gcb,228);
      mask TypeOptions t228_QT_dac2_inter_mode: 1x | 2x | 3x | 4x | 5x | 6x | 8x | 10x | 12x | 16x | 20x | 24x | 40x
      mask Callback t228_QT_dac2_inter_mode:
      | % if I/Q output mode, need to copy interp factor before updating axis clk
      | % note only the even slice for the tile makes this check
      | if chk_param(gcb, 't228_QT_dac2_analog_output', 'I/Q')
      |   inter_mode = get_param(gcb, 't228_QT_dac2_inter_mode');
      |   set_param(gcb, 't228_QT_dac3_inter_mode', inter_mode);
      | end
      | update_axis_clk(gcb,228);
      mask TypeOptions t228_QT_dac2_sample_per_cycle: 4 | 5 | 6 | 7 | 8 | 9 | 10 | 11 | 12 | 13 | 14 | 15 | 16
      mask Callback t228_QT_dac2_sample_per_cycle:
      | % if I/Q output mode, need to copy samples per clk before updating axis clk
      | % note only the even slice for the tile makes this check
      | if chk_param(gcb, 't228_QT_dac2_analog_output', 'I/Q')
      |   spc = get_param(gcb, 't228_QT_dac2_sample_per_cycle');
      |   set_param(gcb, 't228_QT_dac3_sample_per_cycle', spc);
      | end
      | update_axis_clk_label(gcb,228);
      mask TypeOptions t228_QT_dac2_datapath_mode: DUC 0 to Fs/2 | DUC 0 to Fs/4 | DUC Fs/4 to Fs/2 | No DUC 0 to Fs/2
      mask TypeOptions t228_QT_dac2_mixer_type: Fine | Coarse
      mask Callback t228_QT_dac2_mixer_type: mixertype_callback(gcb,228,2,'QT');
      mask TypeOptions t228_QT_dac2_mixer_mode: Real -> Real | I/Q -> Real
      mask Callback t228_QT_dac2_mixer_mode: mixer_callback(gcb,228,2,'QT')
      mask TypeOptions t228_QT_dac2_coarse_freq: 0
      mask TypeOptions t228_QT_dac2_nyquist_zone: Zone 1 | Zone 2
      mask TypeOptions t228_QT_dac2_decode_mode: SNR Optimized | Linearity Optimized
      mask Callback t228_QT_dac3_enable: enable_dac_opt(gcb,228,3,'QT');
      mask TypeOptions t228_QT_dac3_analog_output: Real | I/Q
      mask Callback t228_QT_dac3_analog_output:
      | validate_analog_data(gcb,228,3,'QT');
      | update_axis_clk(gcb,228);
      mask TypeOptions t228_QT_dac3_inter_mode: 1x | 2x | 3x | 4x | 5x | 6x | 8x | 10x | 12x | 16x | 20x | 24x | 40x
      mask Callback t228_QT_dac3_inter_mode: update_axis_clk(gcb,228);
      mask TypeOptions t228_QT_dac3_sample_per_cycle: 4 | 5 | 6 | 7 | 8 | 9 | 10 | 11 | 12 | 13 | 14 | 15 | 16
      mask Callback t228_QT_dac3_sample_per_cycle: update_axis_clk_label(gcb,228);
      mask TypeOptions t228_QT_dac3_datapath_mode: DUC 0 to Fs/2 | DUC 0 to Fs/4 | DUC Fs/4 to Fs/2 | No DUC 0 to Fs/2
      mask TypeOptions t228_QT_dac3_mixer_type: Fine | Coarse
      mask Callback t228_QT_dac3_mixer_type: mixertype_callback(gcb,228,3,'QT');
      mask TypeOptions t228_QT_dac3_mixer_mode: Real -> Real | I/Q -> Real
      mask Callback t228_QT_dac3_mixer_mode: mixer_callback(gcb,228,3,'QT')
      mask TypeOptions t228_QT_dac3_coarse_freq: 0
      mask TypeOptions t228_QT_dac3_nyquist_zone: Zone 1 | Zone 2
      mask TypeOptions t228_QT_dac3_decode_mode: SNR Optimized | Linearity Optimized
      mask Callback t228_DT_dac0_enable: enable_dac_opt(gcb,228,0,'DT');
      mask TypeOptions t228_DT_dac0_analog_output: Real | I/Q
      mask Callback t228_DT_dac0_analog_output:
      | validate_analog_data(gcb,228,0,'DT');
      | update_axis_clk(gcb,228);
      mask TypeOptions t228_DT_dac0_inter_mode: 1x | 2x | 3x | 4x | 5x | 6x | 8x | 10x | 12x | 16x | 20x | 24x | 40x
      mask Callback t228_DT_dac0_inter_mode:
      | % if I/Q output mode, need to copy interp factor before updating axis clk
      | % note only the even slice for the tile makes this check
      | if chk_param(gcb, 't228_DT_dac0_analog_output', 'I/Q')
      |   inter_mode = get_param(gcb, 't228_DT_dac0_inter_mode');
      |   set_param(gcb, 't228_DT_dac1_inter_mode', inter_mode);
      | end
      | 
      | update_axis_clk(gcb,228);
      mask TypeOptions t228_DT_dac0_sample_per_cycle: 4 | 5 | 6 | 7 | 8 | 9 | 10 | 11 | 12 | 13 | 14 | 15 | 16
      mask Callback t228_DT_dac0_sample_per_cycle:
      | % if I/Q output mode, need to copy samples per clk before updating axis clk
      | if chk_param(gcb, 't228_DT_dac0_analog_output', 'I/Q')
      |   spc = get_param(gcb, 't228_DT_dac0_sample_per_cycle');
      |   set_param(gcb, 't228_DT_dac1_sample_per_cycle', spc);
      | end
      | update_axis_clk_label(gcb,228);
      mask TypeOptions t228_DT_dac0_mixer_type: Fine | Coarse
      mask Callback t228_DT_dac0_mixer_type: mixertype_callback(gcb,228,0,'DT');
      mask TypeOptions t228_DT_dac0_mixer_mode: Real -> Real | I/Q -> Real
      mask Callback t228_DT_dac0_mixer_mode: mixer_callback(gcb,228,0,'DT');
      mask TypeOptions t228_DT_dac0_coarse_freq: 0
      mask TypeOptions t228_DT_dac0_nyquist_zone: Zone 1 | Zone 2
      mask TypeOptions t228_DT_dac0_decode_mode: SNR Optimized | Linearity Optimized
      mask Callback t228_DT_dac1_enable: enable_dac_opt(gcb,228,1,'DT');
      mask TypeOptions t228_DT_dac1_analog_output: Real
      mask Callback t228_DT_dac1_analog_output:
      | validate_analog_data(gcb,228,1,'DT');
      | update_axis_clk(gcb,228);
      mask TypeOptions t228_DT_dac1_inter_mode: 1x | 2x | 3x | 4x | 5x | 6x | 8x | 10x | 12x | 16x | 20x | 24x | 40x
      mask Callback t228_DT_dac1_inter_mode: update_axis_clk(gcb,228);
      mask TypeOptions t228_DT_dac1_sample_per_cycle: 4 | 5 | 6 | 7 | 8 | 9 | 10 | 11 | 12 | 13 | 14 | 15 | 16
      mask Callback t228_DT_dac1_sample_per_cycle:
      | %update_axis_clk(gcb);
      | update_axis_clk_label(gcb,228);
      mask TypeOptions t228_DT_dac1_mixer_type: Fine | Coarse
      mask Callback t228_DT_dac1_mixer_type: mixertype_callback(gcb,228,1,'DT');
      mask TypeOptions t228_DT_dac1_mixer_mode: Real -> Real | I/Q -> Real
      mask Callback t228_DT_dac1_mixer_mode: mixer_callback(gcb,228,1,'DT');
      mask TypeOptions t228_DT_dac1_coarse_freq: 0
      mask TypeOptions t228_DT_dac1_nyquist_zone: Zone 1 | Zone 2
      mask TypeOptions t228_DT_dac1_decode_mode: SNR Optimized | Linearity Optimized
      mask Callback t229_sample_rate: update_rfdc_clocking(gcb,229);
      mask TypeOptions t229_clk_out: 125 | 62.5 | 31.25 | 15.625
      mask Callback t229_enable_pll:
      | %update_rfdc_clocking(gcb);
      | update_pll(gcb,229);
      mask TypeOptions t229_ref_clk: 2000
      mask Callback t229_QT_dac0_enable: enable_dac_opt(gcb,229,0,'QT');
      mask TypeOptions t229_QT_dac0_analog_output: Real | I/Q
      mask Callback t229_QT_dac0_analog_output:
      | validate_analog_data(gcb,229,0,'QT');
      | update_axis_clk(gcb,229);
      mask TypeOptions t229_QT_dac0_inter_mode: 1x | 2x | 3x | 4x | 5x | 6x | 8x | 10x | 12x | 16x | 20x | 24x | 40x
      mask Callback t229_QT_dac0_inter_mode:
      | % if I/Q output mode, need to copy interp factor before updating axis clk
      | % note only the even slice for the tile makes this check
      | if chk_param(gcb, 't229_QT_dac0_analog_output', 'I/Q')
      |   inter_mode = get_param(gcb, 't229_QT_dac0_inter_mode');
      |   set_param(gcb, 't229_QT_dac1_inter_mode', inter_mode);
      | end
      | update_axis_clk(gcb,229);
      mask TypeOptions t229_QT_dac0_sample_per_cycle: 4 | 5 | 6 | 7 | 8 | 9 | 10 | 11 | 12 | 13 | 14 | 15 | 16
      mask Callback t229_QT_dac0_sample_per_cycle:
      | % if I/Q output mode, need to copy samples per clk before updating axis clk
      | % note only the even slice for the tile makes this check
      | if chk_param(gcb, 't229_QT_dac0_analog_output', 'I/Q')
      |   spc = get_param(gcb, 't229_QT_dac0_sample_per_cycle');
      |   set_param(gcb, 't229_QT_dac1_sample_per_cycle', spc);
      | end
      | update_axis_clk_label(gcb,229);
      mask TypeOptions t229_QT_dac0_datapath_mode: DUC 0 to Fs/2 | DUC 0 to Fs/4 | DUC Fs/4 to Fs/2 | No DUC 0 to Fs/2
      mask TypeOptions t229_QT_dac0_mixer_type: Fine | Coarse
      mask Callback t229_QT_dac0_mixer_type: mixertype_callback(gcb,229,0,'QT');
      mask TypeOptions t229_QT_dac0_mixer_mode: Real -> Real | I/Q -> Real
      mask Callback t229_QT_dac0_mixer_mode: mixer_callback(gcb,229,0,'QT');
      mask TypeOptions t229_QT_dac0_coarse_freq: 0
      mask TypeOptions t229_QT_dac0_nyquist_zone: Zone 1 | Zone 2
      mask TypeOptions t229_QT_dac0_decode_mode: SNR Optimized | Linearity Optimized
      mask Callback t229_QT_dac1_enable: enable_dac_opt(gcb,229,1,'QT');
      mask TypeOptions t229_QT_dac1_analog_output: Real
      mask Callback t229_QT_dac1_analog_output:
      | validate_analog_data(gcb,229,1,'QT');
      | update_axis_clk(gcb,229);
      mask TypeOptions t229_QT_dac1_inter_mode: 1x | 2x | 3x | 4x | 5x | 6x | 8x | 10x | 12x | 16x | 20x | 24x | 40x
      mask Callback t229_QT_dac1_inter_mode: update_axis_clk(gcb,229);
      mask TypeOptions t229_QT_dac1_sample_per_cycle: 4 | 5 | 6 | 7 | 8 | 9 | 10 | 11 | 12 | 13 | 14 | 15 | 16
      mask Callback t229_QT_dac1_sample_per_cycle: update_axis_clk_label(gcb,229);
      mask TypeOptions t229_QT_dac1_datapath_mode: DUC 0 to Fs/2 | DUC 0 to Fs/4 | DUC Fs/4 to Fs/2 | No DUC 0 to Fs/2
      mask TypeOptions t229_QT_dac1_mixer_type: Fine | Coarse
      mask Callback t229_QT_dac1_mixer_type: mixertype_callback(gcb,229,1,'QT');
      mask TypeOptions t229_QT_dac1_mixer_mode: Real -> Real | I/Q -> Real
      mask Callback t229_QT_dac1_mixer_mode: mixer_callback(gcb,229,1,'QT')
      mask TypeOptions t229_QT_dac1_coarse_freq: 0
      mask TypeOptions t229_QT_dac1_nyquist_zone: Zone 1 | Zone 2
      mask TypeOptions t229_QT_dac1_decode_mode: SNR Optimized | Linearity Optimized
      mask Callback t229_QT_dac2_enable: enable_dac_opt(gcb,229,2,'QT');
      mask TypeOptions t229_QT_dac2_analog_output: Real | I/Q
      mask Callback t229_QT_dac2_analog_output:
      | validate_analog_data(gcb,229,2,'QT');
      | update_axis_clk(gcb,229);
      mask TypeOptions t229_QT_dac2_inter_mode: 1x | 2x | 3x | 4x | 5x | 6x | 8x | 10x | 12x | 16x | 20x | 24x | 40x
      mask Callback t229_QT_dac2_inter_mode:
      | % if I/Q output mode, need to copy interp factor before updating axis clk
      | % note only the even slice for the tile makes this check
      | if chk_param(gcb, 't229_QT_dac2_analog_output', 'I/Q')
      |   inter_mode = get_param(gcb, 't229_QT_dac2_inter_mode');
      |   set_param(gcb, 't229_QT_dac3_inter_mode', inter_mode);
      | end
      | update_axis_clk(gcb,229);
      mask TypeOptions t229_QT_dac2_sample_per_cycle: 4 | 5 | 6 | 7 | 8 | 9 | 10 | 11 | 12 | 13 | 14 | 15 | 16
      mask Callback t229_QT_dac2_sample_per_cycle:
      | % if I/Q output mode, need to copy samples per clk before updating axis clk
      | % note only the even slice for the tile makes this check
      | if chk_param(gcb, 't229_QT_dac2_analog_output', 'I/Q')
      |   spc = get_param(gcb, 't229_QT_dac2_sample_per_cycle');
      |   set_param(gcb, 't229_QT_dac3_sample_per_cycle', spc);
      | end
      | update_axis_clk_label(gcb,229);
      mask TypeOptions t229_QT_dac2_datapath_mode: DUC 0 to Fs/2 | DUC 0 to Fs/4 | DUC Fs/4 to Fs/2 | No DUC 0 to Fs/2
      mask TypeOptions t229_QT_dac2_mixer_type: Fine | Coarse
      mask Callback t229_QT_dac2_mixer_type: mixertype_callback(gcb,229,2,'QT');
      mask TypeOptions t229_QT_dac2_mixer_mode: Real -> Real | I/Q -> Real
      mask Callback t229_QT_dac2_mixer_mode: mixer_callback(gcb,229,2,'QT')
      mask TypeOptions t229_QT_dac2_coarse_freq: 0
      mask TypeOptions t229_QT_dac2_nyquist_zone: Zone 1 | Zone 2
      mask TypeOptions t229_QT_dac2_decode_mode: SNR Optimized | Linearity Optimized
      mask Callback t229_QT_dac3_enable: enable_dac_opt(gcb,229,3,'QT');
      mask TypeOptions t229_QT_dac3_analog_output: Real | I/Q
      mask Callback t229_QT_dac3_analog_output:
      | validate_analog_data(gcb,229,3,'QT');
      | update_axis_clk(gcb,229);
      mask TypeOptions t229_QT_dac3_inter_mode: 1x | 2x | 3x | 4x | 5x | 6x | 8x | 10x | 12x | 16x | 20x | 24x | 40x
      mask Callback t229_QT_dac3_inter_mode: update_axis_clk(gcb,229);
      mask TypeOptions t229_QT_dac3_sample_per_cycle: 4 | 5 | 6 | 7 | 8 | 9 | 10 | 11 | 12 | 13 | 14 | 15 | 16
      mask Callback t229_QT_dac3_sample_per_cycle: update_axis_clk_label(gcb,229);
      mask TypeOptions t229_QT_dac3_datapath_mode: DUC 0 to Fs/2 | DUC 0 to Fs/4 | DUC Fs/4 to Fs/2 | No DUC 0 to Fs/2
      mask TypeOptions t229_QT_dac3_mixer_type: Fine | Coarse
      mask Callback t229_QT_dac3_mixer_type: mixertype_callback(gcb,229,3,'QT');
      mask TypeOptions t229_QT_dac3_mixer_mode: Real -> Real | I/Q -> Real
      mask Callback t229_QT_dac3_mixer_mode: mixer_callback(gcb,229,3,'QT')
      mask TypeOptions t229_QT_dac3_coarse_freq: 0
      mask TypeOptions t229_QT_dac3_nyquist_zone: Zone 1 | Zone 2
      mask TypeOptions t229_QT_dac3_decode_mode: SNR Optimized | Linearity Optimized
      mask Callback t229_DT_dac0_enable: enable_dac_opt(gcb,229,0,'DT');
      mask TypeOptions t229_DT_dac0_analog_output: Real | I/Q
      mask Callback t229_DT_dac0_analog_output:
      | validate_analog_data(gcb,229,0,'DT');
      | update_axis_clk(gcb,229);
      mask TypeOptions t229_DT_dac0_inter_mode: 1x | 2x | 3x | 4x | 5x | 6x | 8x | 10x | 12x | 16x | 20x | 24x | 40x
      mask Callback t229_DT_dac0_inter_mode:
      | % if I/Q output mode, need to copy interp factor before updating axis clk
      | % note only the even slice for the tile makes this check
      | if chk_param(gcb, 't229_DT_dac0_analog_output', 'I/Q')
      |   inter_mode = get_param(gcb, 't229_DT_dac0_inter_mode');
      |   set_param(gcb, 't229_DT_dac1_inter_mode', inter_mode);
      | end
      | update_axis_clk(gcb,229);
      mask TypeOptions t229_DT_dac0_sample_per_cycle: 4 | 5 | 6 | 7 | 8 | 9 | 10 | 11 | 12 | 13 | 14 | 15 | 16
      mask Callback t229_DT_dac0_sample_per_cycle:
      | % if I/Q output mode, need to copy samples per clk before updating axis clk
      | % note only the even slice for the tile makes this check
      | if chk_param(gcb, 't229_DT_dac0_analog_output', 'I/Q')
      |   spc = get_param(gcb, 't229_DT_dac0_sample_per_cycle');
      |   set_param(gcb, 't229_DT_dac1_sample_per_cycle', spc);
      | end
      | update_axis_clk_label(gcb,229);
      mask TypeOptions t229_DT_dac0_mixer_type: Fine | Coarse
      mask Callback t229_DT_dac0_mixer_type: mixertype_callback(gcb,229,0,'DT');
      mask TypeOptions t229_DT_dac0_mixer_mode: Real -> Real | I/Q -> Real
      mask Callback t229_DT_dac0_mixer_mode: mixer_callback(gcb,229,0,'DT');
      mask TypeOptions t229_DT_dac0_coarse_freq: 0
      mask TypeOptions t229_DT_dac0_nyquist_zone: Zone 1 | Zone 2
      mask TypeOptions t229_DT_dac0_decode_mode: SNR Optimized | Linearity Optimized
      mask Callback t229_DT_dac1_enable: enable_dac_opt(gcb,229,1,'DT');
      mask TypeOptions t229_DT_dac1_analog_output: Real
      mask Callback t229_DT_dac1_analog_output:
      | validate_analog_data(gcb,229,1,'DT');
      | update_axis_clk(gcb,229);
      mask TypeOptions t229_DT_dac1_inter_mode: 1x | 2x | 3x | 4x | 5x | 6x | 8x | 10x | 12x | 16x | 20x | 24x | 40x
      mask Callback t229_DT_dac1_inter_mode: update_axis_clk(gcb,229);
      mask TypeOptions t229_DT_dac1_sample_per_cycle: 4 | 5 | 6 | 7 | 8 | 9 | 10 | 11 | 12 | 13 | 14 | 15 | 16
      mask Callback t229_DT_dac1_sample_per_cycle:
      | %update_axis_clk(gcb);
      | update_axis_clk_label(gcb,229);
      mask TypeOptions t229_DT_dac1_mixer_type: Fine | Coarse
      mask Callback t229_DT_dac1_mixer_type: mixertype_callback(gcb,229,1,'DT');
      mask TypeOptions t229_DT_dac1_mixer_mode: Real -> Real | I/Q -> Real
      mask Callback t229_DT_dac1_mixer_mode: mixer_callback(gcb,229,1,'DT');
      mask TypeOptions t229_DT_dac1_coarse_freq: 0
      mask TypeOptions t229_DT_dac1_nyquist_zone: Zone 1 | Zone 2
      mask TypeOptions t229_DT_dac1_decode_mode: SNR Optimized | Linearity Optimized
      mask Callback t230_sample_rate: update_rfdc_clocking(gcb,230);
      mask TypeOptions t230_clk_out: 125 | 62.5 | 31.25 | 15.625
      mask Callback t230_enable_pll:
      | %update_rfdc_clocking(gcb);
      | update_pll(gcb,230);
      mask TypeOptions t230_ref_clk: 2000
      mask Callback t230_QT_dac0_enable: enable_dac_opt(gcb,230,0,'QT');
      mask TypeOptions t230_QT_dac0_analog_output: Real | I/Q
      mask Callback t230_QT_dac0_analog_output:
      | validate_analog_data(gcb,230,0,'QT');
      | update_axis_clk(gcb,230);
      mask TypeOptions t230_QT_dac0_inter_mode: 1x | 2x | 3x | 4x | 5x | 6x | 8x | 10x | 12x | 16x | 20x | 24x | 40x
      mask Callback t230_QT_dac0_inter_mode:
      | % if I/Q output mode, need to copy interp factor before updating axis clk
      | % note only the even slice for the tile makes this check
      | if chk_param(gcb, 't230_QT_dac0_analog_output', 'I/Q')
      |   inter_mode = get_param(gcb, 't230_QT_dac0_inter_mode');
      |   set_param(gcb, 't230_QT_dac1_inter_mode', inter_mode);
      | end
      | update_axis_clk(gcb,230);
      mask TypeOptions t230_QT_dac0_sample_per_cycle: 4 | 5 | 6 | 7 | 8 | 9 | 10 | 11 | 12 | 13 | 14 | 15 | 16
      mask Callback t230_QT_dac0_sample_per_cycle:
      | % if I/Q output mode, need to copy samples per clk before updating axis clk
      | % note only the even slice for the tile makes this check
      | if chk_param(gcb, 't230_QT_dac0_analog_output', 'I/Q')
      |   spc = get_param(gcb, 't230_QT_dac0_sample_per_cycle');
      |   set_param(gcb, 't230_QT_dac1_sample_per_cycle', spc);
      | end
      | 
      | update_axis_clk_label(gcb,230);
      mask TypeOptions t230_QT_dac0_datapath_mode: DUC 0 to Fs/2 | DUC 0 to Fs/4 | DUC Fs/4 to Fs/2 | No DUC 0 to Fs/2
      mask TypeOptions t230_QT_dac0_mixer_type: Fine | Coarse
      mask Callback t230_QT_dac0_mixer_type: mixertype_callback(gcb,230,0,'QT');
      mask TypeOptions t230_QT_dac0_mixer_mode: Real -> Real | I/Q -> Real
      mask Callback t230_QT_dac0_mixer_mode: mixer_callback(gcb,230,0,'QT');
      mask TypeOptions t230_QT_dac0_coarse_freq: 0
      mask TypeOptions t230_QT_dac0_nyquist_zone: Zone 1 | Zone 2
      mask TypeOptions t230_QT_dac0_decode_mode: SNR Optimized | Linearity Optimized
      mask Callback t230_QT_dac1_enable: enable_dac_opt(gcb,230,1,'QT');
      mask TypeOptions t230_QT_dac1_analog_output: Real | I/Q
      mask Callback t230_QT_dac1_analog_output:
      | validate_analog_data(gcb,230,1,'QT');
      | update_axis_clk(gcb,230);
      mask TypeOptions t230_QT_dac1_inter_mode: 1x | 2x | 3x | 4x | 5x | 6x | 8x | 10x | 12x | 16x | 20x | 24x | 40x
      mask Callback t230_QT_dac1_inter_mode: update_axis_clk(gcb,230);
      mask TypeOptions t230_QT_dac1_sample_per_cycle: 4 | 5 | 6 | 7 | 8 | 9 | 10 | 11 | 12 | 13 | 14 | 15 | 16
      mask Callback t230_QT_dac1_sample_per_cycle: update_axis_clk_label(gcb,230);
      mask TypeOptions t230_QT_dac1_datapath_mode: DUC 0 to Fs/2 | DUC 0 to Fs/4 | DUC Fs/4 to Fs/2 | No DUC 0 to Fs/2
      mask TypeOptions t230_QT_dac1_mixer_type: Fine | Coarse
      mask Callback t230_QT_dac1_mixer_type: mixertype_callback(gcb,230,1,'QT');
      mask TypeOptions t230_QT_dac1_mixer_mode: Real -> Real | I/Q -> Real
      mask Callback t230_QT_dac1_mixer_mode: mixer_callback(gcb,230,1,'QT')
      mask TypeOptions t230_QT_dac1_coarse_freq: 0
      mask TypeOptions t230_QT_dac1_nyquist_zone: Zone 1 | Zone 2
      mask TypeOptions t230_QT_dac1_decode_mode: SNR Optimized | Linearity Optimized
      mask Callback t230_QT_dac2_enable: enable_dac_opt(gcb,230,2,'QT');
      mask TypeOptions t230_QT_dac2_analog_output: Real | I/Q
      mask Callback t230_QT_dac2_analog_output:
      | validate_analog_data(gcb,230,2,'QT');
      | update_axis_clk(gcb,230);
      mask TypeOptions t230_QT_dac2_inter_mode: 1x | 2x | 3x | 4x | 5x | 6x | 8x | 10x | 12x | 16x | 20x | 24x | 40x
      mask Callback t230_QT_dac2_inter_mode:
      | % if I/Q output mode, need to copy interp factor before updating axis clk
      | % note only the even slice for the tile makes this check
      | if chk_param(gcb, 't230_QT_dac2_analog_output', 'I/Q')
      |   inter_mode = get_param(gcb, 't230_QT_dac2_inter_mode');
      |   set_param(gcb, 't230_QT_dac3_inter_mode', inter_mode);
      | end
      | 
      | update_axis_clk(gcb,230);
      mask TypeOptions t230_QT_dac2_sample_per_cycle: 4 | 5 | 6 | 7 | 8 | 9 | 10 | 11 | 12 | 13 | 14 | 15 | 16
      mask Callback t230_QT_dac2_sample_per_cycle:
      | % if I/Q output mode, need to copy samples per clk before updating axis clk
      | % note only the even slice for the tile makes this check
      | if chk_param(gcb, 't230_QT_dac2_analog_output', 'I/Q')
      |   spc = get_param(gcb, 't230_QT_dac2_sample_per_cycle');
      |   set_param(gcb, 't230_QT_dac3_sample_per_cycle', spc);
      | end
      | 
      | update_axis_clk_label(gcb,230)
      mask TypeOptions t230_QT_dac2_datapath_mode: DUC 0 to Fs/2 | DUC 0 to Fs/4 | DUC Fs/4 to Fs/2 | No DUC 0 to Fs/2
      mask TypeOptions t230_QT_dac2_mixer_type: Fine | Coarse
      mask Callback t230_QT_dac2_mixer_type: mixertype_callback(gcb,230,2,'QT');
      mask TypeOptions t230_QT_dac2_mixer_mode: Real -> Real | I/Q -> Real
      mask Callback t230_QT_dac2_mixer_mode: mixer_callback(gcb,230,2,'QT')
      mask TypeOptions t230_QT_dac2_coarse_freq: 0
      mask TypeOptions t230_QT_dac2_nyquist_zone: Zone 1 | Zone 2
      mask TypeOptions t230_QT_dac2_decode_mode: SNR Optimized | Linearity Optimized
      mask Callback t230_QT_dac3_enable: enable_dac_opt(gcb,230,3,'QT');
      mask TypeOptions t230_QT_dac3_analog_output: Real | I/Q
      mask Callback t230_QT_dac3_analog_output:
      | validate_analog_data(gcb,230,3,'QT');
      | update_axis_clk(gcb,230);
      mask TypeOptions t230_QT_dac3_inter_mode: 1x | 2x | 3x | 4x | 5x | 6x | 8x | 10x | 12x | 16x | 20x | 24x | 40x
      mask Callback t230_QT_dac3_inter_mode: update_axis_clk(gcb,230);
      mask TypeOptions t230_QT_dac3_sample_per_cycle: 4 | 5 | 6 | 7 | 8 | 9 | 10 | 11 | 12 | 13 | 14 | 15 | 16
      mask Callback t230_QT_dac3_sample_per_cycle: update_axis_clk_label(gcb,230);
      mask TypeOptions t230_QT_dac3_datapath_mode: DUC 0 to Fs/2 | DUC 0 to Fs/4 | DUC Fs/4 to Fs/2 | No DUC 0 to Fs/2
      mask TypeOptions t230_QT_dac3_mixer_type: Fine | Coarse
      mask Callback t230_QT_dac3_mixer_type: mixertype_callback(gcb,230,3,'QT');
      mask TypeOptions t230_QT_dac3_mixer_mode: Real -> Real | I/Q -> Real
      mask Callback t230_QT_dac3_mixer_mode: mixer_callback(gcb,230,3,'QT')
      mask TypeOptions t230_QT_dac3_coarse_freq: 0
      mask TypeOptions t230_QT_dac3_nyquist_zone: Zone 1 | Zone 2
      mask TypeOptions t230_QT_dac3_decode_mode: SNR Optimized | Linearity Optimized
      mask Callback t230_DT_dac0_enable: enable_dac_opt(gcb,230,0,'DT');
      mask TypeOptions t230_DT_dac0_analog_output: Real | I/Q
      mask Callback t230_DT_dac0_analog_output:
      | validate_analog_data(gcb,230,0,'DT');
      | update_axis_clk(gcb,230);
      mask TypeOptions t230_DT_dac0_inter_mode: 1x | 2x | 3x | 4x | 5x | 6x | 8x | 10x | 12x | 16x | 20x | 24x | 40x
      mask Callback t230_DT_dac0_inter_mode:
      | % if I/Q output mode, need to copy interp factor before updating axis clk
      | % note only the even slice for the tile makes this check
      | if chk_param(gcb, 't230_DT_dac0_analog_output', 'I/Q')
      |   inter_mode = get_param(gcb, 't230_DT_dac0_inter_mode');
      |   set_param(gcb, 't230_DT_dac1_inter_mode', inter_mode);
      | end
      | 
      | update_axis_clk(gcb,230);
      mask TypeOptions t230_DT_dac0_sample_per_cycle: 4 | 5 | 6 | 7 | 8 | 9 | 10 | 11 | 12 | 13 | 14 | 15 | 16
      mask Callback t230_DT_dac0_sample_per_cycle:
      | % if I/Q output mode, need to copy samples per clk before updating axis clk
      | % note only the even slice for the tile makes this check
      | if chk_param(gcb, 't230_DT_dac0_analog_output', 'I/Q')
      |   spc = get_param(gcb, 't230_DT_dac0_sample_per_cycle');
      |   set_param(gcb, 't230_DT_dac1_sample_per_cycle', spc);
      | end
      | update_axis_clk_label(gcb,230);
      mask TypeOptions t230_DT_dac0_mixer_type: Fine | Coarse
      mask Callback t230_DT_dac0_mixer_type: mixertype_callback(gcb,230,0,'DT');
      mask TypeOptions t230_DT_dac0_mixer_mode: Real -> Real | I/Q -> Real
      mask Callback t230_DT_dac0_mixer_mode: mixer_callback(gcb,230,0,'DT');
      mask TypeOptions t230_DT_dac0_coarse_freq: 0
      mask TypeOptions t230_DT_dac0_nyquist_zone: Zone 1 | Zone 2
      mask TypeOptions t230_DT_dac0_decode_mode: SNR Optimized | Linearity Optimized
      mask Callback t230_DT_dac1_enable: enable_dac_opt(gcb,230,1,'DT');
      mask TypeOptions t230_DT_dac1_analog_output: Real
      mask Callback t230_DT_dac1_analog_output:
      | validate_analog_data(gcb,230,1,'DT');
      | update_axis_clk(gcb,229);
      mask TypeOptions t230_DT_dac1_inter_mode: 1x | 2x | 3x | 4x | 5x | 6x | 8x | 10x | 12x | 16x | 20x | 24x | 40x
      mask Callback t230_DT_dac1_inter_mode: update_axis_clk(gcb,230);
      mask TypeOptions t230_DT_dac1_sample_per_cycle: 4 | 5 | 6 | 7 | 8 | 9 | 10 | 11 | 12 | 13 | 14 | 15 | 16
      mask Callback t230_DT_dac1_sample_per_cycle:
      | %update_axis_clk(gcb);
      | update_axis_clk_label(gcb,230);
      mask TypeOptions t230_DT_dac1_mixer_type: Fine | Coarse
      mask Callback t230_DT_dac1_mixer_type: mixertype_callback(gcb,230,1,'DT');
      mask TypeOptions t230_DT_dac1_mixer_mode: Real -> Real | I/Q -> Real
      mask Callback t230_DT_dac1_mixer_mode: mixer_callback(gcb,230,1,'DT');
      mask TypeOptions t230_DT_dac1_coarse_freq: 0
      mask TypeOptions t230_DT_dac1_nyquist_zone: Zone 1 | Zone 2
      mask TypeOptions t230_DT_dac1_decode_mode: SNR Optimized | Linearity Optimized
      mask Callback t231_sample_rate: update_rfdc_clocking(gcb,231);
      mask TypeOptions t231_clk_out: 125 | 62.5 | 31.25 | 15.625
      mask Callback t231_enable_pll:
      | %update_rfdc_clocking(gcb);
      | update_pll(gcb,231);
      mask TypeOptions t231_ref_clk: 2000
      mask Callback t231_QT_dac0_enable: enable_dac_opt(gcb,231,0,'QT');
      mask TypeOptions t231_QT_dac0_analog_output: Real | I/Q
      mask Callback t231_QT_dac0_analog_output:
      | validate_analog_data(gcb,231,0,'QT');
      | update_axis_clk(gcb,231);
      mask TypeOptions t231_QT_dac0_inter_mode: 1x | 2x | 3x | 4x | 5x | 6x | 8x | 10x | 12x | 16x | 20x | 24x | 40x
      mask Callback t231_QT_dac0_inter_mode:
      | % if I/Q output mode, need to copy interp factor before updating axis clk
      | % note only the even slice for the tile makes this check
      | if chk_param(gcb, 't231_QT_dac0_analog_output', 'I/Q')
      |   inter_mode = get_param(gcb, 't231_QT_dac0_inter_mode');
      |   set_param(gcb, 't231_QT_dac1_inter_mode', inter_mode);
      | end
      | update_axis_clk(gcb,231);
      mask TypeOptions t231_QT_dac0_sample_per_cycle: 4 | 5 | 6 | 7 | 8 | 9 | 10 | 11 | 12 | 13 | 14 | 15 | 16
      mask Callback t231_QT_dac0_sample_per_cycle:
      | % if I/Q output mode, need to copy samples per clk before updating axis clk
      | % note only the even slice for the tile makes this check
      | if chk_param(gcb, 't231_QT_dac0_analog_output', 'I/Q')
      |   spc = get_param(gcb, 't231_QT_dac0_sample_per_cycle');
      |   set_param(gcb, 't231_QT_dac1_sample_per_cycle', spc);
      | end
      | update_axis_clk_label(gcb,231);
      mask TypeOptions t231_QT_dac0_datapath_mode: DUC 0 to Fs/2 | DUC 0 to Fs/4 | DUC Fs/4 to Fs/2 | No DUC 0 to Fs/2
      mask TypeOptions t231_QT_dac0_mixer_type: Fine | Coarse
      mask Callback t231_QT_dac0_mixer_type: mixertype_callback(gcb,231,0,'QT');
      mask TypeOptions t231_QT_dac0_mixer_mode: Real -> Real | I/Q -> Real
      mask Callback t231_QT_dac0_mixer_mode: mixer_callback(gcb,231,0,'QT');
      mask TypeOptions t231_QT_dac0_coarse_freq: 0
      mask TypeOptions t231_QT_dac0_nyquist_zone: Zone 1 | Zone 2
      mask TypeOptions t231_QT_dac0_decode_mode: SNR Optimized | Linearity Optimized
      mask Callback t231_QT_dac1_enable: enable_dac_opt(gcb,231,1,'QT');
      mask TypeOptions t231_QT_dac1_analog_output: Real | I/Q
      mask Callback t231_QT_dac1_analog_output:
      | validate_analog_data(gcb,231,1,'QT');
      | update_axis_clk(gcb,231);
      mask TypeOptions t231_QT_dac1_inter_mode: 1x | 2x | 3x | 4x | 5x | 6x | 8x | 10x | 12x | 16x | 20x | 24x | 40x
      mask Callback t231_QT_dac1_inter_mode: update_axis_clk(gcb,231);
      mask TypeOptions t231_QT_dac1_sample_per_cycle: 4 | 5 | 6 | 7 | 8 | 9 | 10 | 11 | 12 | 13 | 14 | 15 | 16
      mask Callback t231_QT_dac1_sample_per_cycle: update_axis_clk_label(gcb,231);
      mask TypeOptions t231_QT_dac1_datapath_mode: DUC 0 to Fs/2 | DUC 0 to Fs/4 | DUC Fs/4 to Fs/2 | No DUC 0 to Fs/2
      mask TypeOptions t231_QT_dac1_mixer_type: Fine | Coarse
      mask Callback t231_QT_dac1_mixer_type: mixertype_callback(gcb,231,1,'QT');
      mask TypeOptions t231_QT_dac1_mixer_mode: Real -> Real | I/Q -> Real
      mask Callback t231_QT_dac1_mixer_mode: mixer_callback(gcb,231,1,'QT')
      mask TypeOptions t231_QT_dac1_coarse_freq: 0
      mask TypeOptions t231_QT_dac1_nyquist_zone: Zone 1 | Zone 2
      mask TypeOptions t231_QT_dac1_decode_mode: SNR Optimized | Linearity Optimized
      mask Callback t231_QT_dac2_enable: enable_dac_opt(gcb,231,2,'QT');
      mask TypeOptions t231_QT_dac2_analog_output: Real | I/Q
      mask Callback t231_QT_dac2_analog_output:
      | validate_analog_data(gcb,231,2,'QT');
      | update_axis_clk(gcb,231);
      mask TypeOptions t231_QT_dac2_inter_mode: 1x | 2x | 3x | 4x | 5x | 6x | 8x | 10x | 12x | 16x | 20x | 24x | 40x
      mask Callback t231_QT_dac2_inter_mode:
      | % if I/Q output mode, need to copy interp factor before updating axis clk
      | % note only the even slice for the tile makes this check
      | if chk_param(gcb, 't231_QT_dac2_analog_output', 'I/Q')
      |   inter_mode = get_param(gcb, 't231_QT_dac2_inter_mode');
      |   set_param(gcb, 't231_QT_dac3_inter_mode', inter_mode);
      | end
      | update_axis_clk(gcb,231);
      mask TypeOptions t231_QT_dac2_sample_per_cycle: 4 | 5 | 6 | 7 | 8 | 9 | 10 | 11 | 12 | 13 | 14 | 15 | 16
      mask Callback t231_QT_dac2_sample_per_cycle:
      | % if I/Q output mode, need to copy samples per clk before updating axis clk
      | % note only the even slice for the tile makes this check
      | if chk_param(gcb, 't231_QT_dac2_analog_output', 'I/Q')
      |   spc = get_param(gcb, 't231_QT_dac2_sample_per_cycle');
      |   set_param(gcb, 't231_QT_dac3_sample_per_cycle', spc);
      | end
      | update_axis_clk_label(gcb,231);
      mask TypeOptions t231_QT_dac2_datapath_mode: DUC 0 to Fs/2 | DUC 0 to Fs/4 | DUC Fs/4 to Fs/2 | No DUC 0 to Fs/2
      mask TypeOptions t231_QT_dac2_mixer_type: Fine | Coarse
      mask Callback t231_QT_dac2_mixer_type: mixertype_callback(gcb,231,2,'QT');
      mask TypeOptions t231_QT_dac2_mixer_mode: Real -> Real | I/Q -> Real
      mask Callback t231_QT_dac2_mixer_mode: mixer_callback(gcb,231,2,'QT')
      mask TypeOptions t231_QT_dac2_coarse_freq: 0
      mask TypeOptions t231_QT_dac2_nyquist_zone: Zone 1 | Zone 2
      mask TypeOptions t231_QT_dac2_decode_mode: SNR Optimized | Linearity Optimized
      mask Callback t231_QT_dac3_enable: enable_dac_opt(gcb,231,3,'QT');
      mask TypeOptions t231_QT_dac3_analog_output: Real | I/Q
      mask Callback t231_QT_dac3_analog_output:
      | validate_analog_data(gcb,231,3,'QT');
      | update_axis_clk(gcb,231);
      mask TypeOptions t231_QT_dac3_inter_mode: 1x | 2x | 3x | 4x | 5x | 6x | 8x | 10x | 12x | 16x | 20x | 24x | 40x
      mask Callback t231_QT_dac3_inter_mode: update_axis_clk(gcb,231);
      mask TypeOptions t231_QT_dac3_sample_per_cycle: 4 | 5 | 6 | 7 | 8 | 9 | 10 | 11 | 12 | 13 | 14 | 15 | 16
      mask Callback t231_QT_dac3_sample_per_cycle: update_axis_clk_label(gcb,231);
      mask TypeOptions t231_QT_dac3_datapath_mode: DUC 0 to Fs/2 | DUC 0 to Fs/4 | DUC Fs/4 to Fs/2 | No DUC 0 to Fs/2
      mask TypeOptions t231_QT_dac3_mixer_type: Fine | Coarse
      mask Callback t231_QT_dac3_mixer_type: mixertype_callback(gcb,231,3,'QT');
      mask TypeOptions t231_QT_dac3_mixer_mode: Real -> Real | I/Q -> Real
      mask Callback t231_QT_dac3_mixer_mode: mixer_callback(gcb,231,3,'QT')
      mask TypeOptions t231_QT_dac3_coarse_freq: 0
      mask TypeOptions t231_QT_dac3_nyquist_zone: Zone 1 | Zone 2
      mask TypeOptions t231_QT_dac3_decode_mode: SNR Optimized | Linearity Optimized
      mask Callback t231_DT_dac0_enable: enable_dac_opt(gcb,231,0,'DT');
      mask TypeOptions t231_DT_dac0_analog_output: Real | I/Q
      mask Callback t231_DT_dac0_analog_output:
      | validate_analog_data(gcb,231,0,'DT');
      | update_axis_clk(gcb,231);
      mask TypeOptions t231_DT_dac0_inter_mode: 1x | 2x | 3x | 4x | 5x | 6x | 8x | 10x | 12x | 16x | 20x | 24x | 40x
      mask Callback t231_DT_dac0_inter_mode:
      | % if I/Q output mode, need to copy interp factor before updating axis clk
      | % note only the even slice for the tile makes this check
      | if chk_param(gcb, 't231_DT_dac0_analog_output', 'I/Q')
      |   inter_mode = get_param(gcb, 't231_DT_dac0_inter_mode');
      |   set_param(gcb, 't231_DT_dac1_inter_mode', inter_mode);
      | end
      | update_axis_clk(gcb,231);
      mask TypeOptions t231_DT_dac0_sample_per_cycle: 4 | 5 | 6 | 7 | 8 | 9 | 10 | 11 | 12 | 13 | 14 | 15 | 16
      mask Callback t231_DT_dac0_sample_per_cycle:
      | % if I/Q output mode, need to copy samples per clk before updating axis clk
      | % note only the even slice for the tile makes this check
      | if chk_param(gcb, 't231_DT_dac0_analog_output', 'I/Q')
      |   spc = get_param(gcb, 't231_DT_dac0_sample_per_cycle');
      |   set_param(gcb, 't231_DT_dac1_sample_per_cycle', spc);
      | end
      | update_axis_clk_label(gcb,231);
      mask TypeOptions t231_DT_dac0_mixer_type: Fine | Coarse
      mask Callback t231_DT_dac0_mixer_type: mixertype_callback(gcb,231,0,'DT');
      mask TypeOptions t231_DT_dac0_mixer_mode: Real -> Real | I/Q -> Real
      mask Callback t231_DT_dac0_mixer_mode: mixer_callback(gcb,231,0,'DT');
      mask TypeOptions t231_DT_dac0_coarse_freq: 0
      mask TypeOptions t231_DT_dac0_nyquist_zone: Zone 1 | Zone 2
      mask TypeOptions t231_DT_dac0_decode_mode: SNR Optimized | Linearity Optimized
      mask Callback t231_DT_dac1_enable: enable_dac_opt(gcb,231,1,'DT');
      mask TypeOptions t231_DT_dac1_analog_output: Real
      mask Callback t231_DT_dac1_analog_output:
      | validate_analog_data(gcb,231,1,'DT');
      | update_axis_clk(gcb,231);
      mask TypeOptions t231_DT_dac1_inter_mode: 1x | 2x | 3x | 4x | 5x | 6x | 8x | 10x | 12x | 16x | 20x | 24x | 40x
      mask Callback t231_DT_dac1_inter_mode: update_axis_clk(gcb,231);
      mask TypeOptions t231_DT_dac1_sample_per_cycle: 4 | 5 | 6 | 7 | 8 | 9 | 10 | 11 | 12 | 13 | 14 | 15 | 16
      mask Callback t231_DT_dac1_sample_per_cycle: update_axis_clk_label(gcb,231);
      mask TypeOptions t231_DT_dac1_mixer_type: Fine | Coarse
      mask Callback t231_DT_dac1_mixer_type: mixertype_callback(gcb,231,1,'DT');
      mask TypeOptions t231_DT_dac1_mixer_mode: Real -> Real | I/Q -> Real
      mask Callback t231_DT_dac1_mixer_mode: mixer_callback(gcb,231,1,'DT');
      mask TypeOptions t231_DT_dac1_coarse_freq: 0
      mask TypeOptions t231_DT_dac1_nyquist_zone: Zone 1 | Zone 2
      mask TypeOptions t231_DT_dac1_decode_mode: SNR Optimized | Linearity Optimized
      mask TypeOptions t224_adc_clk_src: 224 | 225 | 226 | 227 | 228 | 229 | 230 | 231
      mask TypeOptions t224_clk_dist: None | Input Refclk | PLL Output
      mask TypeOptions t225_adc_clk_src: 224 | 225 | 226 | 227 | 228 | 229 | 230 | 231
      mask TypeOptions t225_clk_dist: None | Input Refclk | PLL Output
      mask TypeOptions t226_adc_clk_src: 224 | 225 | 226 | 227 | 228 | 229 | 230 | 231
      mask TypeOptions t226_clk_dist: None | Input Refclk | PLL Output
      mask TypeOptions t227_adc_clk_src: 224 | 225 | 226 | 227 | 228 | 229 | 230 | 231
      mask TypeOptions t227_clk_dist: None | Input Refclk | PLL Output
      mask TypeOptions t228_dac_clk_src: 224 | 225 | 226 | 227 | 228 | 229 | 230 | 231
      mask TypeOptions t228_clk_dist: None | Input Refclk | PLL Output
      mask TypeOptions t229_dac_clk_src: 224 | 225 | 226 | 227 | 228 | 229 | 230 | 231
      mask TypeOptions t229_clk_dist: None | Input Refclk | PLL Output
      mask TypeOptions t230_dac_clk_src: 224 | 225 | 226 | 227 | 228 | 229 | 230 | 231
      mask TypeOptions t230_clk_dist: None | Input Refclk | PLL Output
      mask TypeOptions t231_dac_clk_src: 224 | 225 | 226 | 227 | 228 | 229 | 230 | 231
      mask TypeOptions t231_clk_dist: None | Input Refclk | PLL Output
      mask Callback maskdoneopening:
      | %assignin('base','mask_opening',0)
      | %assignin('base','run_init',1)
      | set_param(gcb,'maskopening','0')
      | set_param(gcb,'runinit','1')
      mask DialogControl ADCTileSelect Prompt: ADC Tiles
      mask DialogControl Tile224_container Prompt: Tile 224
      mask DialogControl pll_clocking_config_224 Prompt: Clocking and PLL Configuration
      mask DialogControl t224_QuadTileConfig Prompt: Quad Tile Configuration
      mask DialogControl t224_ADCPair01 Prompt: ADC Pair 0,1
      mask DialogControl t224_QT_adc0 Prompt: ADC 0
      mask DialogControl t224_QT_adc0_DataSettings Prompt: Data Settings
      mask DialogControl t224_QT_adc0_req_axis_clk_label Prompt: Required AXI4-Stream clock:
      mask DialogControl t224_QT_adc0_MixerSettings Prompt: MIxer Settings
      mask DialogControl t224_QT_adc0_AnalogSettings Prompt: Analog Settings
      mask DialogControl t224_QT_adc1 Prompt: ADC 1
      mask DialogControl t224_QT_adc1_DataSettings Prompt: Data Settings
      mask DialogControl t224_QT_adc1_req_axis_clk_label Prompt: Required AXI4-Stream clock:
      mask DialogControl t224_QT_adc1_MixerSettings Prompt: MIxer Settings
      mask DialogControl t224_QT_adc1_AnalogSettings Prompt: Analog Settings
      mask DialogControl ADCPair23 Prompt: ADC Pair 2,3
      mask DialogControl QT_adc2 Prompt: ADC 2
      mask DialogControl t224_QT_adc2_DataSettings Prompt: Data Settings
      mask DialogControl t224_QT_adc2_req_axis_clk_label Prompt: Required AXI4-Stream clock:
      mask DialogControl t224_QT_adc2_MixerSettings Prompt: MIxer Settings
      mask DialogControl t224_QT_adc2_AnalogSettings Prompt: Analog Settings
      mask DialogControl t224_QT_adc3 Prompt: ADC 3
      mask DialogControl t224_QT_adc3_DataSettings Prompt: Data Settings
      mask DialogControl t224_QT_adc3_req_axis_clk_label Prompt: Required AXI4-Stream clock:
      mask DialogControl t224_QT_adc3_MixerSettings Prompt: MIxer Settings
      mask DialogControl t224_QT_adc3_AnalogSettings Prompt: Analog Settings
      mask DialogControl t224_DualTileConfig Prompt: Dual Tile Configuration
      mask DialogControl t224_DT_adc0 Prompt: ADC 0
      mask DialogControl t224_DT_adc0_DataSettings Prompt: Data Settings
      mask DialogControl t224_DT_adc0_req_axis_clk_label Prompt: Required AXI4-Stream clock:
      mask DialogControl t224_DT_adc0_MixerSettings Prompt: MIxer Settings
      mask DialogControl t224_DT_adc0_AnalogSettings Prompt: Analog Settings
      mask DialogControl t224_DT_adc1 Prompt: ADC 1
      mask DialogControl t224_DT_adc1_DataSettings Prompt: Data Settings
      mask DialogControl t224_DT_adc1_req_axis_clk_label Prompt: Required AXI4-Stream clock:
      mask DialogControl t224_DT_adc1_MixerSettings Prompt: MIxer Settings
      mask DialogControl t224_DT_adc1_AnalogSettings Prompt: Analog Settings
      mask DialogControl Tile225_container Prompt: Tile 225
      mask DialogControl pll_clocking_config_225 Prompt: Clocking and PLL Configuration
      mask DialogControl t225_QuadTileConfig Prompt: Quad Tile Configuration
      mask DialogControl t225_ADCPair01 Prompt: ADC Pair 0,1
      mask DialogControl t225_QT_adc0 Prompt: ADC 0
      mask DialogControl t225_QT_adc0_DataSettings Prompt: Data Settings
      mask DialogControl t225_QT_adc0_req_axis_clk_label Prompt: Required AXI4-Stream clock:
      mask DialogControl t225_QT_adc0_MixerSettings Prompt: MIxer Settings
      mask DialogControl t225_QT_adc0_AnalogSettings Prompt: Analog Settings
      mask DialogControl t225_QT_adc1 Prompt: ADC 1
      mask DialogControl t225_QT_adc1_DataSettings Prompt: Data Settings
      mask DialogControl t225_QT_adc1_req_axis_clk_label Prompt: Required AXI4-Stream clock:
      mask DialogControl t225_QT_adc1_MixerSettings Prompt: MIxer Settings
      mask DialogControl t225_QT_adc1_AnalogSettings Prompt: Analog Settings
      mask DialogControl t225_ADCPair23 Prompt: ADC Pair 2,3
      mask DialogControl t225_QT_adc2 Prompt: ADC 2
      mask DialogControl t225_QT_adc2_DataSettings Prompt: Data Settings
      mask DialogControl t225_QT_adc2_req_axis_clk_label Prompt: Required AXI4-Stream clock:
      mask DialogControl t225_QT_adc2_MixerSettings Prompt: MIxer Settings
      mask DialogControl t225_QT_adc2_AnalogSettings Prompt: Analog Settings
      mask DialogControl t225_QT_adc3 Prompt: ADC 3
      mask DialogControl t225_QT_adc3_DataSettings Prompt: Data Settings
      mask DialogControl t225_QT_adc3_req_axis_clk_label Prompt: Required AXI4-Stream clock:
      mask DialogControl t225_QT_adc3_MixerSettings Prompt: MIxer Settings
      mask DialogControl t225_QT_adc3_AnalogSettings Prompt: Analog Settings
      mask DialogControl t225_DualTileConfig Prompt: Dual Tile Configuration
      mask DialogControl t225_DT_adc0 Prompt: ADC 0
      mask DialogControl t225_DT_adc0_DataSettings Prompt: Data Settings
      mask DialogControl t225_DT_adc0_req_axis_clk_label Prompt: Required AXI4-Stream clock:
      mask DialogControl t225_DT_adc0_MixerSettings Prompt: MIxer Settings
      mask DialogControl t225_DT_adc0_AnalogSettings Prompt: Analog Settings
      mask DialogControl t225_DT_adc1 Prompt: ADC 1
      mask DialogControl t225_DT_adc1_DataSettings Prompt: Data Settings
      mask DialogControl t225_DT_adc1_req_axis_clk_label Prompt: Required AXI4-Stream clock:
      mask DialogControl t225_DT_adc1_MixerSettings Prompt: MIxer Settings
      mask DialogControl t225_DT_adc1_AnalogSettings Prompt: Analog Settings
      mask DialogControl Tile226_container Prompt: Tile 226
      mask DialogControl pll_clocking_config_226 Prompt: Clocking and PLL Configuration
      mask DialogControl t226_QuadTileConfig Prompt: Quad Tile Configuration
      mask DialogControl t226_ADCPair01 Prompt: ADC Pair 0,1
      mask DialogControl t226_QT_adc0 Prompt: ADC 0
      mask DialogControl t226_QT_adc0_DataSettings Prompt: Data Settings
      mask DialogControl t226_QT_adc0_req_axis_clk_label Prompt: Required AXI4-Stream clock:
      mask DialogControl t226_QT_adc0_MixerSettings Prompt: MIxer Settings
      mask DialogControl t226_QT_adc0_AnalogSettings Prompt: Analog Settings
      mask DialogControl t226_QT_adc1 Prompt: ADC 1
      mask DialogControl t226_QT_adc1_DataSettings Prompt: Data Settings
      mask DialogControl t226_QT_adc1_req_axis_clk_label Prompt: Required AXI4-Stream clock:
      mask DialogControl t226_QT_adc1_MixerSettings Prompt: MIxer Settings
      mask DialogControl t226_QT_adc1_AnalogSettings Prompt: Analog Settings
      mask DialogControl t226_ADCPair23 Prompt: ADC Pair 2,3
      mask DialogControl t226_QT_adc2 Prompt: ADC 2
      mask DialogControl t226_QT_adc2_DataSettings Prompt: Data Settings
      mask DialogControl t226_QT_adc2_req_axis_clk_label Prompt: Required AXI4-Stream clock:
      mask DialogControl t226_QT_adc2_MixerSettings Prompt: MIxer Settings
      mask DialogControl t226_QT_adc2_AnalogSettings Prompt: Analog Settings
      mask DialogControl t226_QT_adc3 Prompt: ADC 3
      mask DialogControl t226_QT_adc3_DataSettings Prompt: Data Settings
      mask DialogControl t226_QT_adc3_req_axis_clk_label Prompt: Required AXI4-Stream clock:
      mask DialogControl t226_QT_adc3_MixerSettings Prompt: MIxer Settings
      mask DialogControl t226_QT_adc3_AnalogSettings Prompt: Analog Settings
      mask DialogControl t226_DualTileConfig Prompt: Dual Tile Configuration
      mask DialogControl t226_DT_adc0 Prompt: ADC 0
      mask DialogControl t226_DT_adc0_DataSettings Prompt: Data Settings
      mask DialogControl t226_DT_adc0_req_axis_clk_label Prompt: Required AXI4-Stream clock:
      mask DialogControl t226_DT_adc0_MixerSettings Prompt: MIxer Settings
      mask DialogControl t226_DT_adc0_AnalogSettings Prompt: Analog Settings
      mask DialogControl t226_DT_adc1 Prompt: ADC 1
      mask DialogControl t226_DT_adc1_DataSettings Prompt: Data Settings
      mask DialogControl t226_DT_adc1_req_axis_clk_label Prompt: Required AXI4-Stream clock:
      mask DialogControl t226_DT_adc1_MixerSettings Prompt: MIxer Settings
      mask DialogControl t226_DT_adc1_AnalogSettings Prompt: Analog Settings
      mask DialogControl Tile227_container Prompt: Tile 227
      mask DialogControl pll_clocking_config_227 Prompt: Clocking and PLL Configuration
      mask DialogControl t227_QuadTileConfig Prompt: Quad Tile Configuration
      mask DialogControl t227_ADCPair01 Prompt: ADC Pair 0,1
      mask DialogControl t227_QT_adc0 Prompt: ADC 0
      mask DialogControl t227_QT_adc0_DataSettings Prompt: Data Settings
      mask DialogControl t227_QT_adc0_req_axis_clk_label Prompt: Required AXI4-Stream clock:
      mask DialogControl t227_QT_adc0_MixerSettings Prompt: MIxer Settings
      mask DialogControl t227_QT_adc0_AnalogSettings Prompt: Analog Settings
      mask DialogControl t227_QT_adc1 Prompt: ADC 1
      mask DialogControl t227_QT_adc1_DataSettings Prompt: Data Settings
      mask DialogControl t227_QT_adc1_req_axis_clk_label Prompt: Required AXI4-Stream clock:
      mask DialogControl t227_QT_adc1_MixerSettings Prompt: MIxer Settings
      mask DialogControl t227_QT_adc1_AnalogSettings Prompt: Analog Settings
      mask DialogControl t227_ADCPair23 Prompt: ADC Pair 2,3
      mask DialogControl t227_QT_adc2 Prompt: ADC 2
      mask DialogControl t227_QT_adc2_DataSettings Prompt: Data Settings
      mask DialogControl t227_QT_adc2_req_axis_clk_label Prompt: Required AXI4-Stream clock:
      mask DialogControl t227_QT_adc2_MixerSettings Prompt: MIxer Settings
      mask DialogControl t227_QT_adc2_AnalogSettings Prompt: Analog Settings
      mask DialogControl t227_QT_adc3 Prompt: ADC 3
      mask DialogControl t227_QT_adc3_DataSettings Prompt: Data Settings
      mask DialogControl t227_QT_adc3_req_axis_clk_label Prompt: Required AXI4-Stream clock:
      mask DialogControl t227_QT_adc3_MixerSettings Prompt: MIxer Settings
      mask DialogControl t227_QT_adc3_AnalogSettings Prompt: Analog Settings
      mask DialogControl t227_DualTileConfig Prompt: Dual Tile Configuration
      mask DialogControl t227_DT_adc0 Prompt: ADC 0
      mask DialogControl t227_DT_adc0_DataSettings Prompt: Data Settings
      mask DialogControl t227_DT_adc0_req_axis_clk_label Prompt: Required AXI4-Stream clock:
      mask DialogControl t227_DT_adc0_MixerSettings Prompt: MIxer Settings
      mask DialogControl t227_DT_adc0_AnalogSettings Prompt: Analog Settings
      mask DialogControl t227_DT_adc1 Prompt: ADC 1
      mask DialogControl t227_DT_adc1_DataSettings Prompt: Data Settings
      mask DialogControl t227_DT_adc1_req_axis_clk_label Prompt: Required AXI4-Stream clock:
      mask DialogControl t227_DT_adc1_MixerSettings Prompt: MIxer Settings
      mask DialogControl t227_DT_adc1_AnalogSettings Prompt: Analog Settings
      mask DialogControl DACTileSelect Prompt: DAC Tiles
      mask DialogControl Tile228_container Prompt: Tile 228
      mask DialogControl pll_clocking_config_228 Prompt: Clocking and PLL Configuration
      mask DialogControl t228_QuadTileConfig Prompt: Quad Tile Configuration
      mask DialogControl t228_DACPair01 Prompt: DAC Pair 0,1
      mask DialogControl t228_QT_dac0 Prompt: DAC 0
      mask DialogControl t228_QT_dac0_DataSettings Prompt: Data Settings
      mask DialogControl t228_QT_dac0_req_axis_clk_label Prompt: Required AXI4-Stream clock:
      mask DialogControl t228_QT_dac0_MixerSettings Prompt: MIxer Settings
      mask DialogControl t228_QT_dac0_AnalogSettings Prompt: Analog Settings
      mask DialogControl t228_QT_dac1 Prompt: DAC 1
      mask DialogControl t228_QT_dac1_DataSettings Prompt: Data Settings
      mask DialogControl t228_QT_dac1_req_axis_clk_label Prompt: Required AXI4-Stream clock:
      mask DialogControl t228_QT_dac1_MixerSettings Prompt: MIxer Settings
      mask DialogControl t228_QT_dac1_AnalogSettings Prompt: Analog Settings
      mask DialogControl t228_DACPair23 Prompt: DAC Pair 2,3
      mask DialogControl t228_QT_dac2 Prompt: DAC 2
      mask DialogControl t228_QT_dac2_DataSettings Prompt: Data Settings
      mask DialogControl t228_QT_dac2_req_axis_clk_label Prompt: Required AXI4-Stream clock:
      mask DialogControl t228_QT_dac2_MixerSettings Prompt: MIxer Settings
      mask DialogControl t228_QT_dac2_AnalogSettings Prompt: Analog Settings
      mask DialogControl t228_QT_dac3 Prompt: DAC 3
      mask DialogControl t228_QT_dac3_DataSettings Prompt: Data Settings
      mask DialogControl t228_QT_dac3_req_axis_clk_label Prompt: Required AXI4-Stream clock:
      mask DialogControl t228_QT_dac3_MixerSettings Prompt: MIxer Settings
      mask DialogControl t228_QT_dac3_AnalogSettings Prompt: Analog Settings
      mask DialogControl t228_DualTileConfig Prompt: Dual Tile Configuration
      mask DialogControl t228_DT_dac0 Prompt: DAC 0
      mask DialogControl t228_DT_dac0_DataSettings Prompt: Data Settings
      mask DialogControl t228_DT_dac0_req_axis_clk_label Prompt: Required AXI4-Stream clock:
      mask DialogControl t228_DT_dac0_MixerSettings Prompt: MIxer Settings
      mask DialogControl t228_DT_dac0_AnalogSettings Prompt: Analog Settings
      mask DialogControl t228_DT_dac1 Prompt: DAC 1
      mask DialogControl t228_DT_dac1_DataSettings Prompt: Data Settings
      mask DialogControl t228_DT_dac1_req_axis_clk_label Prompt: Required AXI4-Stream clock:
      mask DialogControl t228_DT_dac1_MixerSettings Prompt: MIxer Settings
      mask DialogControl t228_DT_dac1_AnalogSettings Prompt: Analog Settings
      mask DialogControl Tile229_container Prompt: Tile 229
      mask DialogControl pll_clocking_config_229 Prompt: Clocking and PLL Configuration
      mask DialogControl t229_QuadTileConfig Prompt: Quad Tile Configuration
      mask DialogControl t229_DACPair01 Prompt: DAC Pair 0,1
      mask DialogControl t229_QT_dac0 Prompt: DAC 0
      mask DialogControl t229_QT_dac0_DataSettings Prompt: Data Settings
      mask DialogControl t229_QT_dac0_req_axis_clk_label Prompt: Required AXI4-Stream clock:
      mask DialogControl t229_QT_dac0_MixerSettings Prompt: MIxer Settings
      mask DialogControl t229_QT_dac0_AnalogSettings Prompt: Analog Settings
      mask DialogControl t229_QT_dac1 Prompt: DAC 1
      mask DialogControl t229_QT_dac1_DataSettings Prompt: Data Settings
      mask DialogControl t229_QT_dac1_req_axis_clk_label Prompt: Required AXI4-Stream clock:
      mask DialogControl t229_QT_dac1_MixerSettings Prompt: MIxer Settings
      mask DialogControl t229_QT_dac1_AnalogSettings Prompt: Analog Settings
      mask DialogControl t229_DACPair23 Prompt: DAC Pair 2,3
      mask DialogControl t229_QT_dac2 Prompt: DAC 2
      mask DialogControl t229_QT_dac2_DataSettings Prompt: Data Settings
      mask DialogControl t229_QT_dac2_req_axis_clk_label Prompt: Required AXI4-Stream clock:
      mask DialogControl t229_QT_dac2_MixerSettings Prompt: MIxer Settings
      mask DialogControl t229_QT_dac2_AnalogSettings Prompt: Analog Settings
      mask DialogControl t229_QT_dac3 Prompt: DAC 3
      mask DialogControl t229_QT_dac3_DataSettings Prompt: Data Settings
      mask DialogControl t229_QT_dac3_req_axis_clk_label Prompt: Required AXI4-Stream clock:
      mask DialogControl t229_QT_dac3_MixerSettings Prompt: MIxer Settings
      mask DialogControl t229_QT_dac3_AnalogSettings Prompt: Analog Settings
      mask DialogControl t229_DualTileConfig Prompt: Dual Tile Configuration
      mask DialogControl t229_DT_dac0 Prompt: DAC 0
      mask DialogControl t229_DT_dac0_DataSettings Prompt: Data Settings
      mask DialogControl t229_DT_dac0_req_axis_clk_label Prompt: Required AXI4-Stream clock:
      mask DialogControl t229_DT_dac0_MixerSettings Prompt: MIxer Settings
      mask DialogControl t229_DT_dac0_AnalogSettings Prompt: Analog Settings
      mask DialogControl t229_DT_dac1 Prompt: DAC 1
      mask DialogControl t229_DT_dac1_DataSettings Prompt: Data Settings
      mask DialogControl t229_DT_dac1_req_axis_clk_label Prompt: Required AXI4-Stream clock:
      mask DialogControl t229_DT_dac1_MixerSettings Prompt: MIxer Settings
      mask DialogControl t229_DT_dac1_AnalogSettings Prompt: Analog Settings
      mask DialogControl Tile230_container Prompt: Tile 230
      mask DialogControl pll_clocking_config_230 Prompt: Clocking and PLL Configuration
      mask DialogControl t230_QuadTileConfig Prompt: Quad Tile Configuration
      mask DialogControl t230_DACPair01 Prompt: DAC Pair 0,1
      mask DialogControl t230_QT_dac0 Prompt: DAC 0
      mask DialogControl t230_QT_dac0_DataSettings Prompt: Data Settings
      mask DialogControl t230_QT_dac0_req_axis_clk_label Prompt: Required AXI4-Stream clock:
      mask DialogControl t230_QT_dac0_MixerSettings Prompt: MIxer Settings
      mask DialogControl t230_QT_dac0_AnalogSettings Prompt: Analog Settings
      mask DialogControl t230_QT_dac1 Prompt: DAC 1
      mask DialogControl t230_QT_dac1_DataSettings Prompt: Data Settings
      mask DialogControl t230_QT_dac1_req_axis_clk_label Prompt: Required AXI4-Stream clock:
      mask DialogControl t230_QT_dac1_MixerSettings Prompt: MIxer Settings
      mask DialogControl t230_QT_dac1_AnalogSettings Prompt: Analog Settings
      mask DialogControl t230_DACPair23 Prompt: DAC Pair 2,3
      mask DialogControl t230_QT_dac2 Prompt: DAC 2
      mask DialogControl t230_QT_dac2_DataSettings Prompt: Data Settings
      mask DialogControl t230_QT_dac2_req_axis_clk_label Prompt: Required AXI4-Stream clock:
      mask DialogControl t230_QT_dac2_MixerSettings Prompt: MIxer Settings
      mask DialogControl t230_QT_dac2_AnalogSettings Prompt: Analog Settings
      mask DialogControl t230_QT_dac3 Prompt: DAC 3
      mask DialogControl t230_QT_dac3_DataSettings Prompt: Data Settings
      mask DialogControl t230_QT_dac3_req_axis_clk_label Prompt: Required AXI4-Stream clock:
      mask DialogControl t230_QT_dac3_MixerSettings Prompt: MIxer Settings
      mask DialogControl t230_QT_dac3_AnalogSettings Prompt: Analog Settings
      mask DialogControl t230_DualTileConfig Prompt: Dual Tile Configuration
      mask DialogControl t230_DT_dac0 Prompt: DAC 0
      mask DialogControl t230_DT_dac0_DataSettings Prompt: Data Settings
      mask DialogControl t230_DT_dac0_req_axis_clk_label Prompt: Required AXI4-Stream clock:
      mask DialogControl t230_DT_dac0_MixerSettings Prompt: MIxer Settings
      mask DialogControl t230_DT_dac0_AnalogSettings Prompt: Analog Settings
      mask DialogControl t230_DT_dac1 Prompt: DAC 1
      mask DialogControl t230_DT_dac1_DataSettings Prompt: Data Settings
      mask DialogControl t230_DT_dac1_req_axis_clk_label Prompt: Required AXI4-Stream clock:
      mask DialogControl t230_DT_dac1_MixerSettings Prompt: MIxer Settings
      mask DialogControl t230_DT_dac1_AnalogSettings Prompt: Analog Settings
      mask DialogControl Tile231_container Prompt: Tile 231
      mask DialogControl pll_clocking_config_231 Prompt: Clocking and PLL Configuration
      mask DialogControl t231_QuadTileConfig Prompt: Quad Tile Configuration
      mask DialogControl t231_DACPair01 Prompt: DAC Pair 0,1
      mask DialogControl t231_QT_dac0 Prompt: DAC 0
      mask DialogControl t231_QT_dac0_DataSettings Prompt: Data Settings
      mask DialogControl t231_QT_dac0_req_axis_clk_label Prompt: Required AXI4-Stream clock:
      mask DialogControl t231_QT_dac0_MixerSettings Prompt: MIxer Settings
      mask DialogControl t231_QT_dac0_AnalogSettings Prompt: Analog Settings
      mask DialogControl t231_QT_dac1 Prompt: DAC 1
      mask DialogControl t231_QT_dac1_DataSettings Prompt: Data Settings
      mask DialogControl t231_QT_dac1_req_axis_clk_label Prompt: Required AXI4-Stream clock:
      mask DialogControl t231_QT_dac1_MixerSettings Prompt: MIxer Settings
      mask DialogControl t231_QT_dac1_AnalogSettings Prompt: Analog Settings
      mask DialogControl t231_DACPair23 Prompt: DAC Pair 2,3
      mask DialogControl t231_QT_dac2 Prompt: DAC 2
      mask DialogControl t231_QT_dac2_DataSettings Prompt: Data Settings
      mask DialogControl t231_QT_dac2_req_axis_clk_label Prompt: Required AXI4-Stream clock:
      mask DialogControl t231_QT_dac2_MixerSettings Prompt: MIxer Settings
      mask DialogControl t231_QT_dac2_AnalogSettings Prompt: Analog Settings
      mask DialogControl t231_QT_dac3 Prompt: DAC 3
      mask DialogControl t231_QT_dac3_DataSettings Prompt: Data Settings
      mask DialogControl t231_QT_dac3_req_axis_clk_label Prompt: Required AXI4-Stream clock:
      mask DialogControl t231_QT_dac3_MixerSettings Prompt: MIxer Settings
      mask DialogControl t231_QT_dac3_AnalogSettings Prompt: Analog Settings
      mask DialogControl t231_DualTileConfig Prompt: Dual Tile Configuration
      mask DialogControl t231_DT_dac0 Prompt: DAC 0
      mask DialogControl t231_DT_dac0_DataSettings Prompt: Data Settings
      mask DialogControl t231_DT_dac0_req_axis_clk_label Prompt: Required AXI4-Stream clock:
      mask DialogControl t231_DT_dac0_MixerSettings Prompt: MIxer Settings
      mask DialogControl t231_DT_dac0_AnalogSettings Prompt: Analog Settings
      mask DialogControl t231_DT_dac1 Prompt: DAC 1
      mask DialogControl t231_DT_dac1_DataSettings Prompt: Data Settings
      mask DialogControl t231_DT_dac1_req_axis_clk_label Prompt: Required AXI4-Stream clock:
      mask DialogControl t231_DT_dac1_MixerSettings Prompt: MIxer Settings
      mask DialogControl t231_DT_dac1_AnalogSettings Prompt: Analog Settings
      mask DialogControl SystemClocking Prompt: System Clocking
      mask DialogControl ADCClocking Prompt: ADC Tile Clocking
      mask DialogControl t224_clock_config Prompt: ADC Tile 224
      mask DialogControl t225_clock_config Prompt: ADC Tile 225
      mask DialogControl t226_clock_config Prompt: ADC Tile 226
      mask DialogControl t227_clock_config Prompt: ADC Tile 227
      mask DialogControl DACClocking Prompt: DAC Tile Clocking
      mask DialogControl t228_clock_config Prompt: DAC Tile 228
      mask DialogControl t229_clock_config Prompt: DAC Tile 229
      mask DialogControl t230_clock_config Prompt: DAC Tile 230
      mask DialogControl t231_clock_config Prompt: DAC Tile 231
  simple_bram_vacc10 : Subsystem  AncestorBlock=casper_library_accumulators/simple_bram_vacc  mask(simple_bram_vacc){vec_len=8192, arith_type=Unsigned, n_bits=64, bin_pt=34}
      mask prompts: vec_len "Vector length:"; arith_type "Output type:"; n_bits "Bit width (output):"; bin_pt "Binary point (output):"
      mask help: This simple vector accumulator is based on a shift register. It outputs its previous accumulated vector after a new_acc pulse is received.
      mask init:
      | simple_bram_vacc_init(gcb, ...
      |     'vec_len', vec_len, ...
      |     'arith_type', arith_type, ...
      |     'n_bits', n_bits, ...
      |     'bin_pt', bin_pt);
      mask TypeOptions arith_type: Signed | Unsigned
  simple_bram_vacc11 : Subsystem  AncestorBlock=casper_library_accumulators/simple_bram_vacc  mask(simple_bram_vacc){vec_len=8192, arith_type=Unsigned, n_bits=64, bin_pt=34}
      mask prompts: vec_len "Vector length:"; arith_type "Output type:"; n_bits "Bit width (output):"; bin_pt "Binary point (output):"
      mask help: This simple vector accumulator is based on a shift register. It outputs its previous accumulated vector after a new_acc pulse is received.
      mask init:
      | simple_bram_vacc_init(gcb, ...
      |     'vec_len', vec_len, ...
      |     'arith_type', arith_type, ...
      |     'n_bits', n_bits, ...
      |     'bin_pt', bin_pt);
      mask TypeOptions arith_type: Signed | Unsigned
  simple_bram_vacc12 : Subsystem  AncestorBlock=casper_library_accumulators/simple_bram_vacc  mask(simple_bram_vacc){vec_len=8192, arith_type=Unsigned, n_bits=64, bin_pt=34}
      mask prompts: vec_len "Vector length:"; arith_type "Output type:"; n_bits "Bit width (output):"; bin_pt "Binary point (output):"
      mask help: This simple vector accumulator is based on a shift register. It outputs its previous accumulated vector after a new_acc pulse is received.
      mask init:
      | simple_bram_vacc_init(gcb, ...
      |     'vec_len', vec_len, ...
      |     'arith_type', arith_type, ...
      |     'n_bits', n_bits, ...
      |     'bin_pt', bin_pt);
      mask TypeOptions arith_type: Signed | Unsigned
  simple_bram_vacc13 : Subsystem  AncestorBlock=casper_library_accumulators/simple_bram_vacc  mask(simple_bram_vacc){vec_len=8192, arith_type=Unsigned, n_bits=64, bin_pt=34}
      mask prompts: vec_len "Vector length:"; arith_type "Output type:"; n_bits "Bit width (output):"; bin_pt "Binary point (output):"
      mask help: This simple vector accumulator is based on a shift register. It outputs its previous accumulated vector after a new_acc pulse is received.
      mask init:
      | simple_bram_vacc_init(gcb, ...
      |     'vec_len', vec_len, ...
      |     'arith_type', arith_type, ...
      |     'n_bits', n_bits, ...
      |     'bin_pt', bin_pt);
      mask TypeOptions arith_type: Signed | Unsigned
  simple_bram_vacc14 : Subsystem  AncestorBlock=casper_library_accumulators/simple_bram_vacc  mask(simple_bram_vacc){vec_len=8192, arith_type=Unsigned, n_bits=64, bin_pt=34}
      mask prompts: vec_len "Vector length:"; arith_type "Output type:"; n_bits "Bit width (output):"; bin_pt "Binary point (output):"
      mask help: This simple vector accumulator is based on a shift register. It outputs its previous accumulated vector after a new_acc pulse is received.
      mask init:
      | simple_bram_vacc_init(gcb, ...
      |     'vec_len', vec_len, ...
      |     'arith_type', arith_type, ...
      |     'n_bits', n_bits, ...
      |     'bin_pt', bin_pt);
      mask TypeOptions arith_type: Signed | Unsigned
  simple_bram_vacc15 : Subsystem  AncestorBlock=casper_library_accumulators/simple_bram_vacc  mask(simple_bram_vacc){vec_len=8192, arith_type=Unsigned, n_bits=64, bin_pt=34}
      mask prompts: vec_len "Vector length:"; arith_type "Output type:"; n_bits "Bit width (output):"; bin_pt "Binary point (output):"
      mask help: This simple vector accumulator is based on a shift register. It outputs its previous accumulated vector after a new_acc pulse is received.
      mask init:
      | simple_bram_vacc_init(gcb, ...
      |     'vec_len', vec_len, ...
      |     'arith_type', arith_type, ...
      |     'n_bits', n_bits, ...
      |     'bin_pt', bin_pt);
      mask TypeOptions arith_type: Signed | Unsigned
  simple_bram_vacc8 : Subsystem  AncestorBlock=casper_library_accumulators/simple_bram_vacc  mask(simple_bram_vacc){vec_len=8192, arith_type=Unsigned, n_bits=64, bin_pt=34}
      mask prompts: vec_len "Vector length:"; arith_type "Output type:"; n_bits "Bit width (output):"; bin_pt "Binary point (output):"
      mask help: This simple vector accumulator is based on a shift register. It outputs its previous accumulated vector after a new_acc pulse is received.
      mask init:
      | simple_bram_vacc_init(gcb, ...
      |     'vec_len', vec_len, ...
      |     'arith_type', arith_type, ...
      |     'n_bits', n_bits, ...
      |     'bin_pt', bin_pt);
      mask TypeOptions arith_type: Signed | Unsigned
  simple_bram_vacc9 : Subsystem  AncestorBlock=casper_library_accumulators/simple_bram_vacc  mask(simple_bram_vacc){vec_len=8192, arith_type=Unsigned, n_bits=64, bin_pt=34}
      mask prompts: vec_len "Vector length:"; arith_type "Output type:"; n_bits "Bit width (output):"; bin_pt "Binary point (output):"
      mask help: This simple vector accumulator is based on a shift register. It outputs its previous accumulated vector after a new_acc pulse is received.
      mask init:
      | simple_bram_vacc_init(gcb, ...
      |     'vec_len', vec_len, ...
      |     'arith_type', arith_type, ...
      |     'n_bits', n_bits, ...
      |     'bin_pt', bin_pt);
      mask TypeOptions arith_type: Signed | Unsigned
  spect_cnt2 : xbsIndex_r4/Counter  cnt_type=Free Running  cnt_to=Inf  operation=Up  start_count=0  cnt_by_val=1  arith_type=Unsigned  n_bits=13  bin_pt=0  load_pin=off  rst=on  en=on  explicit_period=on  period=1  use_behavioral_HDL=off  implementation=Fabric  use_rpm=off  dbl_ovrd=off  block_type=counter
  sync_cnt : Subsystem  Tag=xps:sw_reg  AncestorBlock=xps_library/Memory/software_register  mask(swreg){io_dir=To Processor, io_delay=0, init_val=0, sample_period=1, names=reg, bitwidths=32, bin_pts=0, arith_types=0, sim_port=on, show_format=off}
      mask prompts: io_dir "I/O direction"; io_delay "I/O delay"; init_val "Initial Value"; sample_period "Sample period"; names "Bitfield names [msb...lsb]"; bitwidths "Bitfield widths"; bin_pts "Bitfield binary pts"; arith_types "Bitfield types, ufix=0, fix=1, bool=2"; sim_port "Provide sim input/output?"; show_format "Print format string?"
      mask help: A 32-bit software-accessible register. Can be divided into bitfields of varying widths and types using the fields in the block mask.
      mask init:
      | swreg_init(gcb)
      settings: AttributesFormatString=1output
      mask TypeOptions io_dir: To Processor | From Processor
      mask Callback io_dir:
      | mask_enables = get_param(gcb, 'MaskEnables');
      | mask_names = get_param(gcb, 'MaskNames');
      | if strcmp(get_param(gcb, 'io_dir'), 'To Processor'),
      |     mask_enables{ismember(mask_names, 'sample_period')} = 'off';
      | else
      |     mask_enables{ismember(mask_names, 'sample_period')} = 'on';
      | end
      | set_param(gcb, 'MaskEnables', mask_enables);
      mask DialogControl ParameterTabVar0 Prompt: Setup
  sync_cntr : xbsIndex_r4/Counter  cnt_type=Free Running  cnt_to=Inf  operation=Up  start_count=0  cnt_by_val=1  arith_type=Unsigned  n_bits=32  bin_pt=0  load_pin=off  rst=on  en=on  explicit_period=on  period=1  use_behavioral_HDL=off  implementation=Fabric  use_rpm=off  dbl_ovrd=off  block_type=counter
  sync_gen : Subsystem  AncestorBlock=casper_library_misc/sync_gen  mask(sync_gen){sim_acc_len=1, fft_size=256, fft_simult_inputs=16, pfb_fir_taps=8, reorder_vec=[2  2  4], scale=256}
      mask prompts: sim_acc_len "Simulation Accumulation Length"; fft_size "FFT Size"; fft_simult_inputs "Simultaneous Inputs (FFT)"; pfb_fir_taps "Taps in pfb_fir (use 1 if no pfb_fir)"; reorder_vec "Reorder Orders (e.g. [2 2 2])"
      mask help:
      | This block computes the sync period based on system parameters as
      | described in Casper memo.  Detailed descritions of the block's
      | variables can be found in the 'Block Documentation' section of
      | the CASPER wiki.
      mask init:
      | sync_gen_init(gcb, ...
      |     'sim_acc_len', sim_acc_len, ...
      |     'fft_size', fft_size, ...
      |     'fft_simult_inputs', fft_simult_inputs,...
      |     'pfb_fir_taps', pfb_fir_taps, ...
      |     'reorder_vec', reorder_vec, ...
      |     'scale', scale);
      settings: AttributesFormatString=sim_sync_period=131072
      mask Help:
      | SyncPeriod=LCM(reorder_vec)*(acc_num)*(pfb_fir_len)*(fft_size/fft_simult_inputs)
      | 
      | See CASPER sync pulse memo for more details.
  wires:
  rfdc/3(m10_axis_tdata) -> Terminator1/1
  bus_expand1/4(out5) -> bus_create/4(in4)
  rfdc/2(m02_axis_tdata) -> Mux/3
  bus_expand1/7(out2) -> bus_create/7(in7)
  Mux/1 -> bus_expand1/1(bus_in)
  bus_expand1/1(msb_out8) -> bus_create/1(in1)
  rfdc/8(m32_axis_tdata) -> Terminator3/1
  bus_expand1/2(out7) -> bus_create/2(in2)
  rfdc/5(m20_axis_tdata) -> Mux/4
  rfdc/7(m30_axis_tdata) -> Terminator2/1
  rfdc/4(m12_axis_tdata) -> Terminator11/1
  rfdc/6(m22_axis_tdata) -> Mux/5
  bus_expand1/3(out6) -> bus_create/3(in3)
  bus_expand1/5(out4) -> bus_create/5(in5)
  bus_create/1(bus_out) -> [current_data]
  rfdc/1(m00_axis_tdata) -> Mux/2
  bus_expand1/6(out3) -> bus_create/6(in6)
  bus_expand1/8(lsb_out1) -> bus_create/8(in8)
  [adc_chan_sel] -> Mux/1
  Constant/1 -> adc_chan_sel/1(sim_1)
  adc_chan_sel/1(in_reg) -> [adc_chan_sel]
  sync_gen/1(sync_out) -> Delay33/1
  Delay33/1 -> [sync_gen]
  [pff_in] -> munge1/1(din)
  munge1/1(dout) -> bus_expand/1(bus_in)
  bus_expand/1(msb_out16) -> pfb_fir_real7/2(pol1_in1)
  bus_expand/2(out15) -> pfb_fir_real7/3(pol1_in2)
  bus_expand/3(out14) -> pfb_fir_real7/4(pol1_in3)
  bus_expand/4(out13) -> pfb_fir_real7/5(pol1_in4)
  bus_expand/5(out12) -> pfb_fir_real7/6(pol1_in5)
  bus_expand/6(out11) -> pfb_fir_real7/7(pol1_in6)
  bus_expand/7(out10) -> pfb_fir_real7/8(pol1_in7)
  bus_expand/8(out9) -> pfb_fir_real7/9(pol1_in8)
  bus_expand/9(out8) -> pfb_fir_real7/10(pol1_in9)
  bus_expand/10(out7) -> pfb_fir_real7/11(pol1_in10)
  bus_expand/11(out6) -> pfb_fir_real7/12(pol1_in11)
  bus_expand/12(out5) -> pfb_fir_real7/13(pol1_in12)
  bus_expand/13(out4) -> pfb_fir_real7/14(pol1_in13)
  bus_expand/14(out3) -> pfb_fir_real7/15(pol1_in14)
  bus_expand/15(out2) -> pfb_fir_real7/16(pol1_in15)
  bus_expand/16(lsb_out1) -> pfb_fir_real7/17(pol1_in16)
  [sync_gen] -> pipeline/1(d)
  pipeline/1(q) -> pfb_fir_real7/1(sync)
  pfb_fir_real7/7(pol1_out6) -> bus_create2/6(in6)
  pfb_fir_real7/16(pol1_out15) -> bus_create2/15(in15)
  pfb_fir_real7/2(pol1_out1) -> bus_create2/1(in1)
  pfb_fir_real7/9(pol1_out8) -> bus_create2/8(in8)
  pfb_fir_real7/17(pol1_out16) -> bus_create2/16(in16)
  pfb_fir_real7/13(pol1_out12) -> bus_create2/12(in12)
  pfb_fir_real7/8(pol1_out7) -> bus_create2/7(in7)
  pfb_fir_real7/14(pol1_out13) -> bus_create2/13(in13)
  pfb_fir_real7/3(pol1_out2) -> bus_create2/2(in2)
  pfb_fir_real7/12(pol1_out11) -> bus_create2/11(in11)
  pfb_fir_real7/5(pol1_out4) -> bus_create2/4(in4)
  pfb_fir_real7/10(pol1_out9) -> bus_create2/9(in9)
  pfb_fir_real7/4(pol1_out3) -> bus_create2/3(in3)
  pfb_fir_real7/6(pol1_out5) -> bus_create2/5(in5)
  pfb_fir_real7/11(pol1_out10) -> bus_create2/10(in10)
  pfb_fir_real7/15(pol1_out14) -> bus_create2/14(in14)
  Relational/1 -> Mux3/1
  [dina2] -> Dual Port RAM6/2
  Delay13/1 -> Relational/1, [write_addr2]
  [pff1_sync] -> Counter13/1
  Constant16/1 -> Dual Port RAM6/3
  Constant21/1 -> AddSub/2
  [write_addr2] -> Dual Port RAM6/1
  Constant19/1 -> Dual Port RAM6/6
  Constant20/1 -> Relational/2
  Dual Port RAM6/1 -> Terminator16/1
  AddSub/1 -> Mux3/3
  Delay15/1 -> Mux3/2
  [pff1_sync] -> Counter15/1
  Counter13/1 -> Delay14/1
  Dual Port RAM6/2 -> [ram2_out]
  Delay14/1 -> Delay15/1, AddSub/1
  [read_addr2] -> Dual Port RAM6/4
  Constant18/1 -> Dual Port RAM6/5
  Mux3/1 -> [read_addr2]
  Counter15/1 -> Delay13/1
  fft_wideband_real/7(out05) -> Delay50/1
  bus_expand3/13(out4) -> fft_wideband_real/15(in012)
  fft_wideband_real/1(sync_out) -> [pfb1_sync]
  Delay1/1 -> [pfb_out1]
  fft_wideband_real/3(out01) -> Delay2/1
  bus_expand3/9(out8) -> fft_wideband_real/11(in08)
  bus_expand3/8(out9) -> fft_wideband_real/10(in07)
  fft_wideband_real/10(of) -> Terminator4/1
  Constant1/1 -> fft_wideband_real/2(shift)
  [ram2_out] -> bus_expand3/1(bus_in)
  bus_expand3/7(out10) -> fft_wideband_real/9(in06)
  Delay16/1 -> fft_wideband_real/1(sync)
  bus_expand3/12(out5) -> fft_wideband_real/14(in011)
  fft_wideband_real/4(out02) -> Delay3/1
  bus_expand3/3(out14) -> fft_wideband_real/5(in02)
  bus_expand3/6(out11) -> fft_wideband_real/8(in05)
  bus_expand3/1(msb_out16) -> fft_wideband_real/3(in00)
  fft_wideband_real/5(out03) -> Delay4/1
  bus_expand3/4(out13) -> fft_wideband_real/6(in03)
  fft_wideband_real/6(out04) -> Delay49/1
  bus_expand3/15(out2) -> fft_wideband_real/17(in014)
  Delay4/1 -> [pfb_out4]
  fft_wideband_real/2(out00) -> Delay1/1
  Delay3/1 -> [pfb_out3]
  bus_expand3/11(out6) -> fft_wideband_real/13(in010)
  Delay58/1 -> [pfb_out8]
  Delay57/1 -> [pfb_out7]
  [pff1_sync] -> Delay16/1
  Delay50/1 -> [pfb_out6]
  bus_expand3/5(out12) -> fft_wideband_real/7(in04)
  Delay2/1 -> [pfb_out2]
  bus_expand3/16(lsb_out1) -> fft_wideband_real/18(in015)
  bus_expand3/2(out15) -> fft_wideband_real/4(in01)
  bus_expand3/10(out7) -> fft_wideband_real/12(in09)
  bus_expand3/14(out3) -> fft_wideband_real/16(in013)
  Delay49/1 -> [pfb_out5]
  fft_wideband_real/8(out06) -> Delay57/1
  fft_wideband_real/9(out07) -> Delay58/1
  Counter17/1 -> AddSub3/1
  AddSub3/1 -> [read_addr3]
  Logical9/1 -> Counter17/2
  AddSub2/1 -> AddSub1/2
  Counter2/1 -> AddSub2/1
  [pfb1_sync] -> Counter1/1
  edge_detect1/1(out) -> Logical2/2
  Slice4/1 -> edge_detect3/1(in)
  Delay60/1 -> AddSub3/2
  Delay59/1 -> AddSub2/2
  [en_ctrl1] -> Logical2/1
  Counter4/1 -> Slice3/1
  Counter14/1 -> Slice5/1
  Slice3/1 -> edge_detect2/1(in)
  [en_ctrl1] -> Logical10/1
  Logical3/1 -> Counter3/2
  [en_ctrl1] -> Logical3/1
  Slice1/1 -> edge_detect1/1(in)
  Counter3/1 -> AddSub1/1
  [pfb1_sync] -> Counter2/1, Counter6/1
  Logical10/1 -> Counter7/2
  Counter18/1 -> Slice4/1
  [en_ctrl1] -> Logical9/1
  Counter1/1 -> Delay59/1
  [pfb1_sync] -> Counter17/1, Counter18/1
  AddSub1/1 -> [write_addr3]
  edge_detect3/1(out) -> Logical9/2
  Slice5/1 -> edge_detect4/1(in)
  Counter6/1 -> Slice1/1
  Logical2/1 -> Counter2/2
  [pfb1_sync] -> Counter3/1, Counter4/1
  Counter7/1 -> [mux_sel]
  Counter16/1 -> Delay60/1
  edge_detect2/1(out) -> Logical3/2
  edge_detect4/1(out) -> Logical10/2
  [pfb1_sync] -> Counter16/1
  [pfb1_sync] -> Counter7/1, Counter14/1
  [pfb_out4] -> Dual Port RAM13/2
  Constant17/1 -> Dual Port RAM4/6
  [pfb_out6] -> Dual Port RAM2/2
  Dual Port RAM3/1 -> Terminator30/1
  Dual Port RAM14/1 -> Terminator33/1
  Constant46/1 -> Dual Port RAM3/5
  [read_addr3] -> Dual Port RAM11/4
  Constant28/1 -> Dual Port RAM13/3
  Constant41/1 -> Dual Port RAM2/5
  Constant10/1 -> Dual Port RAM4/3
  [write_addr3] -> Dual Port RAM14/1
  [read_addr3] -> Dual Port RAM3/4
  Constant50/1 -> Dual Port RAM1/6
  [read_addr3] -> Dual Port RAM4/4
  Dual Port RAM4/1 -> Terminator31/1
  [read_addr3] -> Dual Port RAM14/4
  [write_addr3] -> Dual Port RAM1/1
  Dual Port RAM12/1 -> Terminator29/1
  Dual Port RAM3/2 -> [ram3_out2]
  Constant9/1 -> Dual Port RAM2/3
  Constant38/1 -> Dual Port RAM12/3
  Dual Port RAM2/2 -> [ram3_out6]
  [pfb_out8] -> Dual Port RAM12/2
  Constant13/1 -> Dual Port RAM4/5
  Dual Port RAM13/2 -> [ram3_out4]
  [read_addr3] -> Dual Port RAM2/4
  Constant47/1 -> Dual Port RAM3/6
  Constant12/1 -> Dual Port RAM11/5
  Constant42/1 -> Dual Port RAM2/6
  [write_addr3] -> Dual Port RAM12/1
  [pfb_out5] -> Dual Port RAM14/2
  Constant29/1 -> Dual Port RAM13/5
  Dual Port RAM13/1 -> Terminator32/1
  Dual Port RAM1/2 -> [ram3_out1]
  [write_addr3] -> Dual Port RAM2/1
  [pfb_out7] -> Dual Port RAM11/2
  Constant11/1 -> Dual Port RAM11/3
  Dual Port RAM11/2 -> [ram3_out7]
  [write_addr3] -> Dual Port RAM13/1
  Constant30/1 -> Dual Port RAM13/6
  Constant8/1 -> Dual Port RAM3/3
  Constant48/1 -> Dual Port RAM1/3
  Constant37/1 -> Dual Port RAM11/6
  [read_addr3] -> Dual Port RAM12/4
  Constant43/1 -> Dual Port RAM14/3
  [pfb_out1] -> Dual Port RAM1/2
  Constant39/1 -> Dual Port RAM12/5
  [read_addr3] -> Dual Port RAM1/4
  Dual Port RAM1/1 -> Terminator18/1
  [pfb_out2] -> Dual Port RAM3/2
  [write_addr3] -> Dual Port RAM11/1
  Dual Port RAM12/2 -> [ram3_out8]
  Constant49/1 -> Dual Port RAM1/5
  [write_addr3] -> Dual Port RAM4/1
  Dual Port RAM2/1 -> Terminator22/1
  Dual Port RAM11/1 -> Terminator23/1
  Constant40/1 -> Dual Port RAM12/6
  Constant44/1 -> Dual Port RAM14/5
  [write_addr3] -> Dual Port RAM3/1
  [pfb_out3] -> Dual Port RAM4/2
  [read_addr3] -> Dual Port RAM13/4
  Dual Port RAM4/2 -> [ram3_out3]
  Dual Port RAM14/2 -> [ram3_out5]
  Constant45/1 -> Dual Port RAM14/6
  [ram3_out6] -> Mux5/7
  [ram3_out3] -> Mux5/4
  [mux_sel] -> Delay61/1
  [ram3_out5] -> Mux5/6
  [ram3_out7] -> Mux5/8
  [ram3_out4] -> Mux5/5
  [ram3_out2] -> Mux5/3
  [ram3_out8] -> Mux5/9
  Mux5/1 -> munge2/1(din)
  [ram3_out1] -> Mux5/2
  Delay61/1 -> Mux5/1
  bus_expand4/5(out4) -> fft1/7(in04)
  bus_expand4/2(out7) -> fft1/4(in01)
  fft1/10(of) -> Terminator38/1
  bus_expand4/7(out2) -> fft1/9(in06)
  Constant51/1 -> fft1/2(shift)
  Delay72/1 -> fft1/1(sync)
  [pfb1_sync] -> Delay72/1
  bus_expand4/8(lsb_out1) -> fft1/10(in07)
  bus_expand4/1(msb_out8) -> fft1/3(in00)
  bus_expand4/6(out3) -> fft1/8(in05)
  bus_expand4/4(out5) -> fft1/6(in03)
  bus_expand4/3(out6) -> fft1/5(in02)
  munge2/1(dout) -> bus_expand4/1(bus_in)
  Delay66/1 -> power10/1
  pipeline68/1(q) -> q3/2(data_in)
  pipeline80/1(q) -> simple_bram_vacc10/1(new_acc)
  fft1/2(out00) -> Delay64/1
  q4/1(data_out) -> Terminator21/1
  Delay88/1 -> Delay89/1
  acc_cntrl2/1(new_acc) -> [new_acc]
  power12/1 -> Delay78/1
  pipeline88/1(q) -> q5/3(we)
  q6/1(data_out) -> Terminator26/1
  pipeline83/1(q) -> pipeline87/1(d)
  pipeline71/1(q) -> q1/1(addr)
  power14/1 -> Delay86/1
  pipeline62/1(q) -> q2/3(we)
  Delay76/1 -> Delay77/1
  q7/1(data_out) -> Terminator27/1
  pipeline85/1(q) -> simple_bram_vacc14/2(din)
  pipeline86/1(q) -> simple_bram_vacc15/1(new_acc)
  pipeline97/1(q) -> q5/1(addr)
  fft1/8(out06) -> Delay82/1
  power11/1 -> Delay74/1
  simple_bram_vacc9/1(dout) -> Reinterpret12/1
  q5/1(data_out) -> Terminator34/1
  simple_bram_vacc14/1(dout) -> Reinterpret14/1
  simple_bram_vacc14/2(valid) -> pipeline88/1(d)
  power16/1 -> Delay83/1
  power13/1 -> Delay84/1
  pipeline92/1(q) -> q6/2(data_in)
  pipeline57/1(q) -> simple_bram_vacc8/2(din)
  Delay78/1 -> pipeline73/1(d)
  pipeline103/1(q) -> pipeline105/1(d)
  Delay64/1 -> Delay75/1
  simple_bram_vacc11/1(dout) -> Reinterpret10/1
  power10/1 -> Delay70/1
  pipeline74/1(q) -> simple_bram_vacc11/1(new_acc)
  pipeline66/1(q) -> q3/3(we)
  Delay79/1 -> Delay87/1
  Delay69/1 -> pipeline64/1(d)
  pipeline73/1(q) -> pipeline75/1(d)
  Delay77/1 -> power12/1
  pipeline58/1(q) -> simple_bram_vacc9/1(new_acc)
  fft1/9(out07) -> Delay88/1
  Delay80/1 -> Delay81/1
  Delay89/1 -> power15/1
  pipeline69/1(q) -> q4/3(we)
  Delay67/1 -> Delay71/1
  pipeline67/1(q) -> q3/1(addr)
  pipeline100/1(q) -> simple_bram_vacc13/1(new_acc)
  [acc_len] -> acc_cntrl2/1(acc_len)
  [new_acc] -> pipeline56/1(d)
  pipeline101/1(q) -> simple_bram_vacc13/2(din)
  Delay62/1 -> Delay73/1
  Delay85/1 -> power14/1
  simple_bram_vacc12/1(dout) -> Reinterpret16/1
  simple_bram_vacc10/2(valid) -> pipeline66/1(d)
  Delay71/1 -> power11/1
  [new_acc] -> pipeline84/1(d)
  power15/1 -> Delay90/1
  [new_acc] -> pipeline58/1(d)
  Reinterpret11/1 -> pipeline82/1(d)
  spect_cnt2/1 -> pipeline67/1(d), pipeline94/1(d), pipeline98/1(d), pipeline90/1(d), pipeline97/1(d), pipeline72/1(d), pipeline63/1(d), pipeline71/1(d)
  q3/1(data_out) -> Terminator20/1
  Delay73/1 -> Delay68/1
  simple_bram_vacc13/1(dout) -> Reinterpret13/1
  pipeline75/1(q) -> simple_bram_vacc11/2(din)
  Reinterpret16/1 -> pipeline95/1(d)
  q2/1(data_out) -> Terminator19/1
  [new_acc] -> pipeline74/1(d)
  pipeline91/1(q) -> pipeline85/1(d)
  pipeline95/1(q) -> q7/2(data_in)
  simple_bram_vacc15/1(dout) -> Reinterpret15/1
  fft1/7(out05) -> Delay80/1
  fft1/3(out01) -> Delay65/1
  simple_bram_vacc8/1(dout) -> Reinterpret11/1
  [new_acc] -> pipeline104/1(d)
  Delay86/1 -> pipeline103/1(d)
  simple_bram_vacc13/2(valid) -> pipeline96/1(d)
  Delay75/1 -> power9/1
  q1/1(data_out) -> Terminator25/1
  Delay84/1 -> pipeline83/1(d)
  Delay90/1 -> pipeline99/1(d)
  pipeline102/1(q) -> q8/2(data_in)
  simple_bram_vacc15/2(valid) -> pipeline89/1(d)
  pipeline87/1(q) -> simple_bram_vacc15/2(din)
  fft1/4(out02) -> Delay67/1
  Delay70/1 -> pipeline54/1(d)
  power9/1 -> Delay69/1
  pipeline64/1(q) -> pipeline57/1(d)
  pipeline84/1(q) -> simple_bram_vacc14/1(new_acc)
  Reinterpret13/1 -> pipeline102/1(d)
  Delay82/1 -> Delay85/1
  Reinterpret14/1 -> pipeline106/1(d)
  pipeline81/1(q) -> simple_bram_vacc10/2(din)
  pipeline104/1(q) -> simple_bram_vacc12/1(new_acc)
  pipeline94/1(q) -> q7/1(addr)
  pipeline89/1(q) -> q6/3(we)
  Reinterpret7/1 -> pipeline68/1(d)
  pipeline76/1(q) -> q4/2(data_in)
  fft1/1(sync_out) -> Delay63/1
  pipeline98/1(q) -> q8/1(addr)
  pipeline82/1(q) -> q1/2(data_in)
  pipeline90/1(q) -> q6/1(addr)
  pipeline106/1(q) -> q5/2(data_in)
  [new_acc] -> pipeline86/1(d)
  Delay68/1 -> acc_cntrl2/2(sync)
  Delay65/1 -> Delay66/1
  pipeline61/1(q) -> q1/3(we)
  pipeline79/1(q) -> pipeline81/1(d)
  Reinterpret12/1 -> pipeline65/1(d)
  Delay87/1 -> power16/1
  q8/1(data_out) -> Terminator28/1
  [new_acc] -> pipeline80/1(d)
  pipeline93/1(q) -> q7/3(we)
  Delay74/1 -> pipeline79/1(d)
  pipeline105/1(q) -> simple_bram_vacc12/2(din)
  pipeline56/1(q) -> simple_bram_vacc8/1(new_acc)
  Delay63/1 -> Delay62/1
  Delay83/1 -> pipeline91/1(d)
  pipeline96/1(q) -> q8/3(we)
  pipeline55/1(q) -> spect_cnt2/1
  pipeline60/1(q) -> simple_bram_vacc9/2(din)
  Reinterpret15/1 -> pipeline92/1(d)
  fft1/6(out04) -> Delay79/1
  pipeline63/1(q) -> q2/1(addr)
  pipeline54/1(q) -> pipeline60/1(d)
  [new_acc] -> pipeline100/1(d)
  pipeline72/1(q) -> q4/1(addr)
  [new_acc] -> pipeline55/1(d)
  [cnt_rst] -> acc_cntrl2/3(rst)
  fft1/5(out03) -> Delay76/1
  Delay81/1 -> power13/1
  simple_bram_vacc11/2(valid) -> pipeline69/1(d)
  simple_bram_vacc8/2(valid) -> pipeline61/1(d), spect_cnt2/2
  simple_bram_vacc10/1(dout) -> Reinterpret7/1
  simple_bram_vacc12/2(valid) -> pipeline93/1(d)
  pipeline99/1(q) -> pipeline101/1(d)
  pipeline65/1(q) -> q2/2(data_in)
  Reinterpret10/1 -> pipeline76/1(d)
  simple_bram_vacc9/2(valid) -> pipeline62/1(d)
  Constant3/1 -> acc_len/1(sim_1)
  [cnt_rst] -> acc_cntr/1
  acc_len/1(in_reg) -> pipeline2/1(d)
  Delay23/1 -> acc_cntr/2
  Delay6/1 -> acc_cnt/1(out_reg)
  sync_cntr/1 -> Delay21/1
  Delay21/1 -> sync_cnt/1(out_reg)
  acc_cnt/1(sim_out_reg) -> Terminator6/1
  acc_cntr/1 -> Delay6/1
  Constant2/1 -> cnt_rst/1(sim_1)
  pipeline2/1(q) -> [acc_len]
  [cnt_rst] -> sync_cntr/1
  cnt_rst/1(in_reg) -> pipeline1/1(d)
  [sync_gen] -> sync_cntr/2
  [new_acc] -> Delay23/1
  pipeline1/1(q) -> [cnt_rst]
  sync_cnt/1(sim_out_reg) -> Terminator7/1
  [pfb1_sync] -> Counter19/1
  Convert2/1 -> [en_ctrl1]
  Counter19/1 -> Convert2/1
  bus_create2/1(bus_out) -> Delay17/1
  pfb_fir_real7/1(sync_out) -> [pff1_sync]
  Delay17/1 -> [dina2]
  [en_ctrl] -> pfb_fir_real7/18(en_ctrl)
  Constant114/1 -> Relational3/2
  Constant111/1 -> Dual Port RAM16/6
  [sync_gen] -> Counter61/1
  Relational3/1 -> [ram_out_sel]
  Delay139/1 -> Relational3/1
  Counter59/1 -> Slice14/1
  Counter58/1 -> AddSub55/1
  Constant113/1 -> Relational2/2
  [en_ctrl] -> Logical12/1
  [c1] -> Mux13/3
  [sync_gen] -> Counter60/1
  [read_addr] -> Dual Port RAM16/4
  Mux14/1 -> [pff_in]
  [write_addr] -> Dual Port RAM16/1
  Delay136/1 -> Concat6/2
  [sync_gen] -> Counter56/1
  Delay138/1 -> Mux13/1, Relational2/1
  Constant110/1 -> Dual Port RAM16/5
  [os_data] -> Dual Port RAM16/2
  Delay137/1 -> AddSub55/2
  Relational2/1 -> [write_en]
  Counter60/1 -> Delay137/1
  Constant112/1 -> Dual Port RAM16/7
  Logical12/1 -> Counter56/2
  Dual Port RAM16/2 -> [ram_outb]
  [current_data] -> Delay136/1
  [ram_out_sel] -> Mux14/1
  AddSub55/1 -> [read_addr]
  edge_detect15/1(out) -> Logical13/2
  [sync_gen] -> Counter58/1, Counter59/1
  Slice14/1 -> edge_detect15/1(in)
  Counter55/1 -> Delay138/1
  [en_ctrl] -> Logical13/1
  [write_en] -> Dual Port RAM16/3
  Constant109/1 -> Mux13/2
  [ram_outb] -> Mux14/3
  [sync_gen] -> Counter57/1
  Convert6/1 -> [en_ctrl]
  Mux13/1 -> [os_data]
  [write_en] -> Logical12/2
  [ram_outa] -> Mux14/2
  [current_data] -> Concat6/1
  Counter56/1 -> [write_addr]
  Concat6/1 -> [c1]
  [sync_gen] -> Counter55/1
  Logical13/1 -> Counter58/2
  Counter61/1 -> Delay139/1
  Dual Port RAM16/1 -> [ram_outa]
  Counter57/1 -> Convert6/1
